simulink model "XTHERM05_reference"  (R2025a)
settings: Solver=daessc  StartTime=0  StopTime=240  MaxStep=1  RelTol=1e-3  AbsTol=1e-3
undefined symbols (not defined in the file): battery_builder_rtmsupport, charge_current_A, charge_step_fraction, charge_step_time_s, coolant_inlet_temperature_K, gcbh, initial_battery_temperature_K
libraries: BatteryPack96S3P_lib x12, fl_lib x8, nesl_utility x5, BatteryCurrentManagement x1, coolingPlateThermal_lib x1
(part 3 of 3)

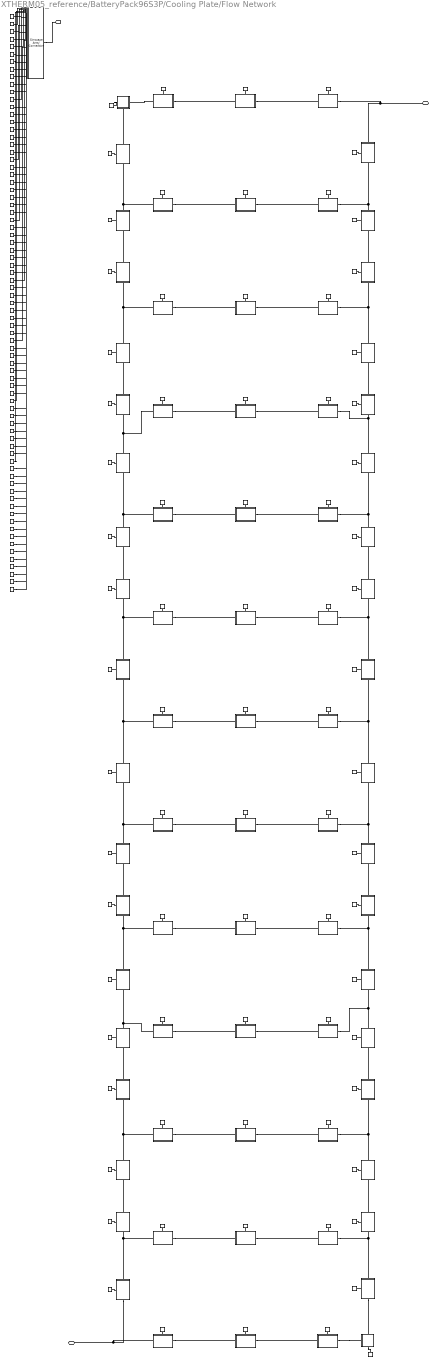
== system XTHERM05_reference/BatteryPack96S3P/Cooling Plate/Flow Network ==
  note: Partition [3,8]
  note: Partition [3,7]
  note: Partition [3,6]
  note: Partition [3,5]
  note: Partition [3,4]
  note: Partition [3,3]
  note: Partition [3,2]
  note: Partition [3,1]
  note: Partition [2,8]
  note: Partition [2,7]
  note: Partition [2,6]
  note: Partition [2,5]
  note: Partition [2,4]
  note: Partition [2,3]
  note: Partition [2,2]
  note: Partition [2,1]
  note: Partition [1,8]
  note: Partition [1,7]
  note: Partition [1,6]
  note: Partition [1,5]
  note: Partition [1,4]
  note: Partition [1,3]
  note: Partition [1,2]
  note: Partition [1,1]
  Array Connection : SimscapeArrayConnection  Domain=foundation.thermal.thermal  NumScalarElements=77
  Bend1_1 : Subsystem  ReferencedSubsystem=BendSubsystemWithMask  lengthPipe=0.0031376  areaPipe=3.1416e-06  diaPipe=0.002  dirPipeOrientBend=up-right
      settings: PortSchema="{\"entries\":[{\"content\":{\"sides\":[{\"content\":{\"connectorIds\":[\"LConn1\"]},\"type\":\"ConnectorPlacement.EquallySpacedRectSide\",\"uuid\":\"fe1e9e2d-1739-4737-8ec3-440461fb646e\"},{\"content\":{\"side\":\"RIGHT\"},\"type\":\"ConnectorPlacement.EquallySpacedRectSide\",\"uuid\":\"c44e4257-eb38-4c5c-b0bd-b7832920e0b4\"},{\"content\":{\"connectorIds\":[\"LConn2\"],\"side\":\"TOP\"},\"type\":\"ConnectorPlacement.EquallySpacedRectSide\",\"uuid\":\"152ce001-782f-4a48-bd0b-9533b0313205\"},{\"content\":{\"connectorIds\":[\"RConn1\"],\"side\":\"BOTTOM\"},\"type\":\"ConnectorPlacement.EquallySpacedRectSide\",\"uuid\":\"9f8ea262-ac4d-418e-a81f-297a07a7dff2\"}]},\"type\":\"ConnectorPlacement.EquallySpacedConnector\",\"uuid\":\"fea8adfe-ce64-4d7f-ba34-bc1e0cac7b5f\"}],\"packageUris\":[\"http://schema.mathworks.com/mf0/Connector/R2020b\"],\"version\":\"1.0\"}"
  Bend2_1 : Subsystem  ReferencedSubsystem=BendSubsystemWithMask  lengthPipe=0.0031376  areaPipe=3.1416e-06  diaPipe=0.002  dirPipeOrientBend=up-right
      settings: PortSchema="{\"entries\":[{\"content\":{\"sides\":[{\"content\":{\"connectorIds\":[\"LConn1\"]},\"type\":\"ConnectorPlacement.EquallySpacedRectSide\",\"uuid\":\"fe1e9e2d-1739-4737-8ec3-440461fb646e\"},{\"content\":{\"side\":\"RIGHT\"},\"type\":\"ConnectorPlacement.EquallySpacedRectSide\",\"uuid\":\"c44e4257-eb38-4c5c-b0bd-b7832920e0b4\"},{\"content\":{\"connectorIds\":[\"LConn2\"],\"side\":\"TOP\"},\"type\":\"ConnectorPlacement.EquallySpacedRectSide\",\"uuid\":\"152ce001-782f-4a48-bd0b-9533b0313205\"},{\"content\":{\"connectorIds\":[\"RConn1\"],\"side\":\"BOTTOM\"},\"type\":\"ConnectorPlacement.EquallySpacedRectSide\",\"uuid\":\"780a4b5e-c251-4558-87ca-52d2b2f91024\"}]},\"type\":\"ConnectorPlacement.EquallySpacedConnector\",\"uuid\":\"fea8adfe-ce64-4d7f-ba34-bc1e0cac7b5f\"}],\"packageUris\":[\"http://schema.mathworks.com/mf0/Connector/R2020b\"],\"version\":\"1.0\"}"
  H_10_1 : ConnectionLabel  Label=H_10_1
  H_10_1_bus : ConnectionLabel  Label=H_10_1
  H_10_2 : ConnectionLabel  Label=H_10_2
  H_10_2_bus : ConnectionLabel  Label=H_10_2
  H_10_3 : ConnectionLabel  Label=H_10_3
  H_10_3_bus : ConnectionLabel  Label=H_10_3
  H_11_1 : ConnectionLabel  Label=H_11_1
  H_11_1_bus : ConnectionLabel  Label=H_11_1
  H_11_2 : ConnectionLabel  Label=H_11_2
  H_11_2_bus : ConnectionLabel  Label=H_11_2
  H_11_3 : ConnectionLabel  Label=H_11_3
  H_11_3_bus : ConnectionLabel  Label=H_11_3
  H_12_1 : ConnectionLabel  Label=H_12_1
  H_12_1_bus : ConnectionLabel  Label=H_12_1
  H_12_2 : ConnectionLabel  Label=H_12_2
  H_12_2_bus : ConnectionLabel  Label=H_12_2
  H_12_3 : ConnectionLabel  Label=H_12_3
  H_12_3_bus : ConnectionLabel  Label=H_12_3
  H_13_1 : ConnectionLabel  Label=H_13_1
  H_13_1_bus : ConnectionLabel  Label=H_13_1
  H_13_2 : ConnectionLabel  Label=H_13_2
  H_13_2_bus : ConnectionLabel  Label=H_13_2
  H_13_3 : ConnectionLabel  Label=H_13_3
  H_13_3_bus : ConnectionLabel  Label=H_13_3
  H_14_1 : ConnectionLabel  Label=H_14_1
  H_14_1_bus : ConnectionLabel  Label=H_14_1
  H_15_1 : ConnectionLabel  Label=H_15_1
  H_15_1_bus : ConnectionLabel  Label=H_15_1
  H_15_2 : ConnectionLabel  Label=H_15_2
  H_15_2_bus : ConnectionLabel  Label=H_15_2
  H_16_1 : ConnectionLabel  Label=H_16_1
  H_16_1_bus : ConnectionLabel  Label=H_16_1
  H_16_2 : ConnectionLabel  Label=H_16_2
  H_16_2_bus : ConnectionLabel  Label=H_16_2
  H_17_1 : ConnectionLabel  Label=H_17_1
  H_17_1_bus : ConnectionLabel  Label=H_17_1
  H_18_1 : ConnectionLabel  Label=H_18_1
  H_18_1_bus : ConnectionLabel  Label=H_18_1
  H_18_2 : ConnectionLabel  Label=H_18_2
  H_18_2_bus : ConnectionLabel  Label=H_18_2
  H_19_1 : ConnectionLabel  Label=H_19_1
  H_19_1_bus : ConnectionLabel  Label=H_19_1
  H_1_1 : ConnectionLabel  Label=H_1_1
  H_1_1_bus : ConnectionLabel  Label=H_1_1
  H_1_2 : ConnectionLabel  Label=H_1_2
  H_1_2_bus : ConnectionLabel  Label=H_1_2
  H_1_3 : ConnectionLabel  Label=H_1_3
  H_1_3_bus : ConnectionLabel  Label=H_1_3
  H_20_1 : ConnectionLabel  Label=H_20_1
  H_20_1_bus : ConnectionLabel  Label=H_20_1
  H_21_1 : ConnectionLabel  Label=H_21_1
  H_21_1_bus : ConnectionLabel  Label=H_21_1
  H_21_2 : ConnectionLabel  Label=H_21_2
  H_21_2_bus : ConnectionLabel  Label=H_21_2
  H_22_1 : ConnectionLabel  Label=H_22_1
  H_22_1_bus : ConnectionLabel  Label=H_22_1
  H_23_1 : ConnectionLabel  Label=H_23_1
  H_23_1_bus : ConnectionLabel  Label=H_23_1
  H_23_2 : ConnectionLabel  Label=H_23_2
  H_23_2_bus : ConnectionLabel  Label=H_23_2
  H_24_1 : ConnectionLabel  Label=H_24_1
  H_24_1_bus : ConnectionLabel  Label=H_24_1
  H_24_2 : ConnectionLabel  Label=H_24_2
  H_24_2_bus : ConnectionLabel  Label=H_24_2
  H_25_1 : ConnectionLabel  Label=H_25_1
  H_25_1_bus : ConnectionLabel  Label=H_25_1
  H_26_1 : ConnectionLabel  Label=H_26_1
  H_26_1_bus : ConnectionLabel  Label=H_26_1
  H_27_1 : ConnectionLabel  Label=H_27_1
  H_27_1_bus : ConnectionLabel  Label=H_27_1
  H_27_2 : ConnectionLabel  Label=H_27_2
  H_27_2_bus : ConnectionLabel  Label=H_27_2
  H_28_1 : ConnectionLabel  Label=H_28_1
  H_28_1_bus : ConnectionLabel  Label=H_28_1
  H_28_2 : ConnectionLabel  Label=H_28_2
  H_28_2_bus : ConnectionLabel  Label=H_28_2
  H_29_1 : ConnectionLabel  Label=H_29_1
  H_29_1_bus : ConnectionLabel  Label=H_29_1
  H_2_1 : ConnectionLabel  Label=H_2_1
  H_2_1_bus : ConnectionLabel  Label=H_2_1
  H_2_2 : ConnectionLabel  Label=H_2_2
  H_2_2_bus : ConnectionLabel  Label=H_2_2
  H_2_3 : ConnectionLabel  Label=H_2_3
  H_2_3_bus : ConnectionLabel  Label=H_2_3
  H_30_1 : ConnectionLabel  Label=H_30_1
  H_30_1_bus : ConnectionLabel  Label=H_30_1
  H_30_2 : ConnectionLabel  Label=H_30_2
  H_30_2_bus : ConnectionLabel  Label=H_30_2
  H_31_1 : ConnectionLabel  Label=H_31_1
  H_31_1_bus : ConnectionLabel  Label=H_31_1
  H_32_1 : ConnectionLabel  Label=H_32_1
  H_32_1_bus : ConnectionLabel  Label=H_32_1
  H_33_1 : ConnectionLabel  Label=H_33_1
  H_33_1_bus : ConnectionLabel  Label=H_33_1
  H_33_2 : ConnectionLabel  Label=H_33_2
  H_33_2_bus : ConnectionLabel  Label=H_33_2
  H_34_1 : ConnectionLabel  Label=H_34_1
  H_34_1_bus : ConnectionLabel  Label=H_34_1
  H_35_1 : ConnectionLabel  Label=H_35_1
  H_35_1_bus : ConnectionLabel  Label=H_35_1
  H_35_2 : ConnectionLabel  Label=H_35_2
  H_35_2_bus : ConnectionLabel  Label=H_35_2
  H_36_1 : ConnectionLabel  Label=H_36_1
  H_36_1_bus : ConnectionLabel  Label=H_36_1
  H_36_2 : ConnectionLabel  Label=H_36_2
  H_36_2_bus : ConnectionLabel  Label=H_36_2
  H_37_1 : ConnectionLabel  Label=H_37_1
  H_37_1_bus : ConnectionLabel  Label=H_37_1
  H_38_1 : ConnectionLabel  Label=H_38_1
  H_38_1_bus : ConnectionLabel  Label=H_38_1
  H_39_1 : ConnectionLabel  Label=H_39_1
  H_39_1_bus : ConnectionLabel  Label=H_39_1
  H_3_1 : ConnectionLabel  Label=H_3_1
  H_3_1_bus : ConnectionLabel  Label=H_3_1
  H_3_2 : ConnectionLabel  Label=H_3_2
  H_3_2_bus : ConnectionLabel  Label=H_3_2
  H_3_3 : ConnectionLabel  Label=H_3_3
  H_3_3_bus : ConnectionLabel  Label=H_3_3
  H_4_1 : ConnectionLabel  Label=H_4_1
  H_4_1_bus : ConnectionLabel  Label=H_4_1
  H_4_2 : ConnectionLabel  Label=H_4_2
  H_4_2_bus : ConnectionLabel  Label=H_4_2
  H_4_3 : ConnectionLabel  Label=H_4_3
  H_4_3_bus : ConnectionLabel  Label=H_4_3
  H_5_1 : ConnectionLabel  Label=H_5_1
  H_5_1_bus : ConnectionLabel  Label=H_5_1
  H_5_2 : ConnectionLabel  Label=H_5_2
  H_5_2_bus : ConnectionLabel  Label=H_5_2
  H_5_3 : ConnectionLabel  Label=H_5_3
  H_5_3_bus : ConnectionLabel  Label=H_5_3
  H_6_1 : ConnectionLabel  Label=H_6_1
  H_6_1_bus : ConnectionLabel  Label=H_6_1
  H_6_2 : ConnectionLabel  Label=H_6_2
  H_6_2_bus : ConnectionLabel  Label=H_6_2
  H_6_3 : ConnectionLabel  Label=H_6_3
  H_6_3_bus : ConnectionLabel  Label=H_6_3
  H_7_1 : ConnectionLabel  Label=H_7_1
  H_7_1_bus : ConnectionLabel  Label=H_7_1
  H_7_2 : ConnectionLabel  Label=H_7_2
  H_7_2_bus : ConnectionLabel  Label=H_7_2
  H_7_3 : ConnectionLabel  Label=H_7_3
  H_7_3_bus : ConnectionLabel  Label=H_7_3
  H_8_1 : ConnectionLabel  Label=H_8_1
  H_8_1_bus : ConnectionLabel  Label=H_8_1
  H_8_2 : ConnectionLabel  Label=H_8_2
  H_8_2_bus : ConnectionLabel  Label=H_8_2
  H_8_3 : ConnectionLabel  Label=H_8_3
  H_8_3_bus : ConnectionLabel  Label=H_8_3
  H_9_1 : ConnectionLabel  Label=H_9_1
  H_9_1_bus : ConnectionLabel  Label=H_9_1
  H_9_2 : ConnectionLabel  Label=H_9_2
  H_9_2_bus : ConnectionLabel  Label=H_9_2
  H_9_3 : ConnectionLabel  Label=H_9_3
  H_9_3_bus : ConnectionLabel  Label=H_9_3
  Pipe10_1 : Subsystem  ReferencedSubsystem=PipeSubsystemWithMask  lengthPipe=0.36667  areaPipe=3.1416e-06  diaPipe=0.002  directionPipe=right
      settings: PortSchema="{\"entries\":[{\"content\":{\"sides\":[{\"content\":{\"connectorIds\":[\"LConn1\"]},\"type\":\"ConnectorPlacement.EquallySpacedRectSide\",\"uuid\":\"fe1e9e2d-1739-4737-8ec3-440461fb646e\"},{\"content\":{\"connectorIds\":[\"RConn1\"],\"side\":\"RIGHT\"},\"type\":\"ConnectorPlacement.EquallySpacedRectSide\",\"uuid\":\"c44e4257-eb38-4c5c-b0bd-b7832920e0b4\"},{\"content\":{\"connectorIds\":[\"LConn2\"],\"side\":\"TOP\"},\"type\":\"ConnectorPlacement.EquallySpacedRectSide\",\"uuid\":\"152ce001-782f-4a48-bd0b-9533b0313205\"}]},\"type\":\"ConnectorPlacement.EquallySpacedConnector\",\"uuid\":\"fea8adfe-ce64-4d7f-ba34-bc1e0cac7b5f\"}],\"packageUris\":[\"http://schema.mathworks.com/mf0/Connector/R2020b\"],\"version\":\"1.0\"}"
  Pipe10_2 : Subsystem  ReferencedSubsystem=PipeSubsystemWithMask  lengthPipe=0.39167  areaPipe=3.1416e-06  diaPipe=0.002  directionPipe=right
      settings: PortSchema="{\"entries\":[{\"content\":{\"sides\":[{\"content\":{\"connectorIds\":[\"LConn1\"]},\"type\":\"ConnectorPlacement.EquallySpacedRectSide\",\"uuid\":\"fe1e9e2d-1739-4737-8ec3-440461fb646e\"},{\"content\":{\"connectorIds\":[\"RConn1\"],\"side\":\"RIGHT\"},\"type\":\"ConnectorPlacement.EquallySpacedRectSide\",\"uuid\":\"c44e4257-eb38-4c5c-b0bd-b7832920e0b4\"},{\"content\":{\"connectorIds\":[\"LConn2\"],\"side\":\"TOP\"},\"type\":\"ConnectorPlacement.EquallySpacedRectSide\",\"uuid\":\"152ce001-782f-4a48-bd0b-9533b0313205\"}]},\"type\":\"ConnectorPlacement.EquallySpacedConnector\",\"uuid\":\"fea8adfe-ce64-4d7f-ba34-bc1e0cac7b5f\"}],\"packageUris\":[\"http://schema.mathworks.com/mf0/Connector/R2020b\"],\"version\":\"1.0\"}"
  Pipe10_3 : Subsystem  ReferencedSubsystem=PipeSubsystemWithMask  lengthPipe=0.36667  areaPipe=3.1416e-06  diaPipe=0.002  directionPipe=right
      settings: PortSchema="{\"entries\":[{\"content\":{\"sides\":[{\"content\":{\"connectorIds\":[\"LConn1\"]},\"type\":\"ConnectorPlacement.EquallySpacedRectSide\",\"uuid\":\"fe1e9e2d-1739-4737-8ec3-440461fb646e\"},{\"content\":{\"connectorIds\":[\"RConn1\"],\"side\":\"RIGHT\"},\"type\":\"ConnectorPlacement.EquallySpacedRectSide\",\"uuid\":\"c44e4257-eb38-4c5c-b0bd-b7832920e0b4\"},{\"content\":{\"connectorIds\":[\"LConn2\"],\"side\":\"TOP\"},\"type\":\"ConnectorPlacement.EquallySpacedRectSide\",\"uuid\":\"152ce001-782f-4a48-bd0b-9533b0313205\"}]},\"type\":\"ConnectorPlacement.EquallySpacedConnector\",\"uuid\":\"fea8adfe-ce64-4d7f-ba34-bc1e0cac7b5f\"}],\"packageUris\":[\"http://schema.mathworks.com/mf0/Connector/R2020b\"],\"version\":\"1.0\"}"
  Pipe11_1 : Subsystem  ReferencedSubsystem=PipeSubsystemWithMask  lengthPipe=0.36667  areaPipe=3.1416e-06  diaPipe=0.002  directionPipe=right
      settings: PortSchema="{\"entries\":[{\"content\":{\"sides\":[{\"content\":{\"connectorIds\":[\"LConn1\"]},\"type\":\"ConnectorPlacement.EquallySpacedRectSide\",\"uuid\":\"fe1e9e2d-1739-4737-8ec3-440461fb646e\"},{\"content\":{\"connectorIds\":[\"RConn1\"],\"side\":\"RIGHT\"},\"type\":\"ConnectorPlacement.EquallySpacedRectSide\",\"uuid\":\"c44e4257-eb38-4c5c-b0bd-b7832920e0b4\"},{\"content\":{\"connectorIds\":[\"LConn2\"],\"side\":\"TOP\"},\"type\":\"ConnectorPlacement.EquallySpacedRectSide\",\"uuid\":\"152ce001-782f-4a48-bd0b-9533b0313205\"}]},\"type\":\"ConnectorPlacement.EquallySpacedConnector\",\"uuid\":\"fea8adfe-ce64-4d7f-ba34-bc1e0cac7b5f\"}],\"packageUris\":[\"http://schema.mathworks.com/mf0/Connector/R2020b\"],\"version\":\"1.0\"}"
  Pipe11_2 : Subsystem  ReferencedSubsystem=PipeSubsystemWithMask  lengthPipe=0.39167  areaPipe=3.1416e-06  diaPipe=0.002  directionPipe=right
      settings: PortSchema="{\"entries\":[{\"content\":{\"sides\":[{\"content\":{\"connectorIds\":[\"LConn1\"]},\"type\":\"ConnectorPlacement.EquallySpacedRectSide\",\"uuid\":\"fe1e9e2d-1739-4737-8ec3-440461fb646e\"},{\"content\":{\"connectorIds\":[\"RConn1\"],\"side\":\"RIGHT\"},\"type\":\"ConnectorPlacement.EquallySpacedRectSide\",\"uuid\":\"c44e4257-eb38-4c5c-b0bd-b7832920e0b4\"},{\"content\":{\"connectorIds\":[\"LConn2\"],\"side\":\"TOP\"},\"type\":\"ConnectorPlacement.EquallySpacedRectSide\",\"uuid\":\"152ce001-782f-4a48-bd0b-9533b0313205\"}]},\"type\":\"ConnectorPlacement.EquallySpacedConnector\",\"uuid\":\"fea8adfe-ce64-4d7f-ba34-bc1e0cac7b5f\"}],\"packageUris\":[\"http://schema.mathworks.com/mf0/Connector/R2020b\"],\"version\":\"1.0\"}"
  Pipe11_3 : Subsystem  ReferencedSubsystem=PipeSubsystemWithMask  lengthPipe=0.36667  areaPipe=3.1416e-06  diaPipe=0.002  directionPipe=right
      settings: PortSchema="{\"entries\":[{\"content\":{\"sides\":[{\"content\":{\"connectorIds\":[\"LConn1\"]},\"type\":\"ConnectorPlacement.EquallySpacedRectSide\",\"uuid\":\"fe1e9e2d-1739-4737-8ec3-440461fb646e\"},{\"content\":{\"connectorIds\":[\"RConn1\"],\"side\":\"RIGHT\"},\"type\":\"ConnectorPlacement.EquallySpacedRectSide\",\"uuid\":\"c44e4257-eb38-4c5c-b0bd-b7832920e0b4\"},{\"content\":{\"connectorIds\":[\"LConn2\"],\"side\":\"TOP\"},\"type\":\"ConnectorPlacement.EquallySpacedRectSide\",\"uuid\":\"152ce001-782f-4a48-bd0b-9533b0313205\"}]},\"type\":\"ConnectorPlacement.EquallySpacedConnector\",\"uuid\":\"fea8adfe-ce64-4d7f-ba34-bc1e0cac7b5f\"}],\"packageUris\":[\"http://schema.mathworks.com/mf0/Connector/R2020b\"],\"version\":\"1.0\"}"
  Pipe12_1 : Subsystem  ReferencedSubsystem=PipeSubsystemWithMask  lengthPipe=0.36667  areaPipe=3.1416e-06  diaPipe=0.002  directionPipe=right
      settings: PortSchema="{\"entries\":[{\"content\":{\"sides\":[{\"content\":{\"connectorIds\":[\"LConn1\"]},\"type\":\"ConnectorPlacement.EquallySpacedRectSide\",\"uuid\":\"fe1e9e2d-1739-4737-8ec3-440461fb646e\"},{\"content\":{\"connectorIds\":[\"RConn1\"],\"side\":\"RIGHT\"},\"type\":\"ConnectorPlacement.EquallySpacedRectSide\",\"uuid\":\"c44e4257-eb38-4c5c-b0bd-b7832920e0b4\"},{\"content\":{\"connectorIds\":[\"LConn2\"],\"side\":\"TOP\"},\"type\":\"ConnectorPlacement.EquallySpacedRectSide\",\"uuid\":\"152ce001-782f-4a48-bd0b-9533b0313205\"}]},\"type\":\"ConnectorPlacement.EquallySpacedConnector\",\"uuid\":\"fea8adfe-ce64-4d7f-ba34-bc1e0cac7b5f\"}],\"packageUris\":[\"http://schema.mathworks.com/mf0/Connector/R2020b\"],\"version\":\"1.0\"}"
  Pipe12_2 : Subsystem  ReferencedSubsystem=PipeSubsystemWithMask  lengthPipe=0.39167  areaPipe=3.1416e-06  diaPipe=0.002  directionPipe=right
      settings: PortSchema="{\"entries\":[{\"content\":{\"sides\":[{\"content\":{\"connectorIds\":[\"LConn1\"]},\"type\":\"ConnectorPlacement.EquallySpacedRectSide\",\"uuid\":\"fe1e9e2d-1739-4737-8ec3-440461fb646e\"},{\"content\":{\"connectorIds\":[\"RConn1\"],\"side\":\"RIGHT\"},\"type\":\"ConnectorPlacement.EquallySpacedRectSide\",\"uuid\":\"c44e4257-eb38-4c5c-b0bd-b7832920e0b4\"},{\"content\":{\"connectorIds\":[\"LConn2\"],\"side\":\"TOP\"},\"type\":\"ConnectorPlacement.EquallySpacedRectSide\",\"uuid\":\"152ce001-782f-4a48-bd0b-9533b0313205\"}]},\"type\":\"ConnectorPlacement.EquallySpacedConnector\",\"uuid\":\"fea8adfe-ce64-4d7f-ba34-bc1e0cac7b5f\"}],\"packageUris\":[\"http://schema.mathworks.com/mf0/Connector/R2020b\"],\"version\":\"1.0\"}"
  Pipe12_3 : Subsystem  ReferencedSubsystem=PipeSubsystemWithMask  lengthPipe=0.36667  areaPipe=3.1416e-06  diaPipe=0.002  directionPipe=right
      settings: PortSchema="{\"entries\":[{\"content\":{\"sides\":[{\"content\":{\"connectorIds\":[\"LConn1\"]},\"type\":\"ConnectorPlacement.EquallySpacedRectSide\",\"uuid\":\"fe1e9e2d-1739-4737-8ec3-440461fb646e\"},{\"content\":{\"connectorIds\":[\"RConn1\"],\"side\":\"RIGHT\"},\"type\":\"ConnectorPlacement.EquallySpacedRectSide\",\"uuid\":\"c44e4257-eb38-4c5c-b0bd-b7832920e0b4\"},{\"content\":{\"connectorIds\":[\"LConn2\"],\"side\":\"TOP\"},\"type\":\"ConnectorPlacement.EquallySpacedRectSide\",\"uuid\":\"152ce001-782f-4a48-bd0b-9533b0313205\"}]},\"type\":\"ConnectorPlacement.EquallySpacedConnector\",\"uuid\":\"fea8adfe-ce64-4d7f-ba34-bc1e0cac7b5f\"}],\"packageUris\":[\"http://schema.mathworks.com/mf0/Connector/R2020b\"],\"version\":\"1.0\"}"
  Pipe13_1 : Subsystem  ReferencedSubsystem=PipeSubsystemWithMask  lengthPipe=0.36467  areaPipe=3.1416e-06  diaPipe=0.002  directionPipe=right
      settings: PortSchema="{\"entries\":[{\"content\":{\"sides\":[{\"content\":{\"connectorIds\":[\"LConn1\"]},\"type\":\"ConnectorPlacement.EquallySpacedRectSide\",\"uuid\":\"fe1e9e2d-1739-4737-8ec3-440461fb646e\"},{\"content\":{\"connectorIds\":[\"RConn1\"],\"side\":\"RIGHT\"},\"type\":\"ConnectorPlacement.EquallySpacedRectSide\",\"uuid\":\"c44e4257-eb38-4c5c-b0bd-b7832920e0b4\"},{\"content\":{\"connectorIds\":[\"LConn2\"],\"side\":\"TOP\"},\"type\":\"ConnectorPlacement.EquallySpacedRectSide\",\"uuid\":\"152ce001-782f-4a48-bd0b-9533b0313205\"}]},\"type\":\"ConnectorPlacement.EquallySpacedConnector\",\"uuid\":\"fea8adfe-ce64-4d7f-ba34-bc1e0cac7b5f\"}],\"packageUris\":[\"http://schema.mathworks.com/mf0/Connector/R2020b\"],\"version\":\"1.0\"}"
  Pipe13_2 : Subsystem  ReferencedSubsystem=PipeSubsystemWithMask  lengthPipe=0.39167  areaPipe=3.1416e-06  diaPipe=0.002  directionPipe=right
      settings: PortSchema="{\"entries\":[{\"content\":{\"sides\":[{\"content\":{\"connectorIds\":[\"LConn1\"]},\"type\":\"ConnectorPlacement.EquallySpacedRectSide\",\"uuid\":\"fe1e9e2d-1739-4737-8ec3-440461fb646e\"},{\"content\":{\"connectorIds\":[\"RConn1\"],\"side\":\"RIGHT\"},\"type\":\"ConnectorPlacement.EquallySpacedRectSide\",\"uuid\":\"c44e4257-eb38-4c5c-b0bd-b7832920e0b4\"},{\"content\":{\"connectorIds\":[\"LConn2\"],\"side\":\"TOP\"},\"type\":\"ConnectorPlacement.EquallySpacedRectSide\",\"uuid\":\"152ce001-782f-4a48-bd0b-9533b0313205\"}]},\"type\":\"ConnectorPlacement.EquallySpacedConnector\",\"uuid\":\"fea8adfe-ce64-4d7f-ba34-bc1e0cac7b5f\"}],\"packageUris\":[\"http://schema.mathworks.com/mf0/Connector/R2020b\"],\"version\":\"1.0\"}"
  Pipe13_3 : Subsystem  ReferencedSubsystem=PipeSubsystemWithMask  lengthPipe=0.36667  areaPipe=3.1416e-06  diaPipe=0.002  directionPipe=right
      settings: PortSchema="{\"entries\":[{\"content\":{\"sides\":[{\"content\":{\"connectorIds\":[\"LConn1\"]},\"type\":\"ConnectorPlacement.EquallySpacedRectSide\",\"uuid\":\"fe1e9e2d-1739-4737-8ec3-440461fb646e\"},{\"content\":{\"connectorIds\":[\"RConn1\"],\"side\":\"RIGHT\"},\"type\":\"ConnectorPlacement.EquallySpacedRectSide\",\"uuid\":\"c44e4257-eb38-4c5c-b0bd-b7832920e0b4\"},{\"content\":{\"connectorIds\":[\"LConn2\"],\"side\":\"TOP\"},\"type\":\"ConnectorPlacement.EquallySpacedRectSide\",\"uuid\":\"152ce001-782f-4a48-bd0b-9533b0313205\"}]},\"type\":\"ConnectorPlacement.EquallySpacedConnector\",\"uuid\":\"fea8adfe-ce64-4d7f-ba34-bc1e0cac7b5f\"}],\"packageUris\":[\"http://schema.mathworks.com/mf0/Connector/R2020b\"],\"version\":\"1.0\"}"
  Pipe14_1 : Subsystem  ReferencedSubsystem=PipeSubsystemWithMask  lengthPipe=0.1  areaPipe=3.1416e-06  diaPipe=0.002  directionPipe=up
      settings: PortSchema="{\"entries\":[{\"content\":{\"sides\":[{\"content\":{\"connectorIds\":[\"LConn1\"]},\"type\":\"ConnectorPlacement.EquallySpacedRectSide\",\"uuid\":\"fe1e9e2d-1739-4737-8ec3-440461fb646e\"},{\"content\":{\"connectorIds\":[\"RConn1\"],\"side\":\"RIGHT\"},\"type\":\"ConnectorPlacement.EquallySpacedRectSide\",\"uuid\":\"c44e4257-eb38-4c5c-b0bd-b7832920e0b4\"},{\"content\":{\"connectorIds\":[\"LConn2\"],\"side\":\"TOP\"},\"type\":\"ConnectorPlacement.EquallySpacedRectSide\",\"uuid\":\"152ce001-782f-4a48-bd0b-9533b0313205\"}]},\"type\":\"ConnectorPlacement.EquallySpacedConnector\",\"uuid\":\"fea8adfe-ce64-4d7f-ba34-bc1e0cac7b5f\"}],\"packageUris\":[\"http://schema.mathworks.com/mf0/Connector/R2020b\"],\"version\":\"1.0\"}"
  Pipe15_1 : Subsystem  ReferencedSubsystem=PipeSubsystemWithMask  lengthPipe=0.03125  areaPipe=3.1416e-06  diaPipe=0.002  directionPipe=up
      settings: PortSchema="{\"entries\":[{\"content\":{\"sides\":[{\"content\":{\"connectorIds\":[\"LConn1\"]},\"type\":\"ConnectorPlacement.EquallySpacedRectSide\",\"uuid\":\"fe1e9e2d-1739-4737-8ec3-440461fb646e\"},{\"content\":{\"connectorIds\":[\"RConn1\"],\"side\":\"RIGHT\"},\"type\":\"ConnectorPlacement.EquallySpacedRectSide\",\"uuid\":\"c44e4257-eb38-4c5c-b0bd-b7832920e0b4\"},{\"content\":{\"connectorIds\":[\"LConn2\"],\"side\":\"TOP\"},\"type\":\"ConnectorPlacement.EquallySpacedRectSide\",\"uuid\":\"152ce001-782f-4a48-bd0b-9533b0313205\"}]},\"type\":\"ConnectorPlacement.EquallySpacedConnector\",\"uuid\":\"fea8adfe-ce64-4d7f-ba34-bc1e0cac7b5f\"}],\"packageUris\":[\"http://schema.mathworks.com/mf0/Connector/R2020b\"],\"version\":\"1.0\"}"
  Pipe15_2 : Subsystem  ReferencedSubsystem=PipeSubsystemWithMask  lengthPipe=0.06875  areaPipe=3.1416e-06  diaPipe=0.002  directionPipe=up
      settings: PortSchema="{\"entries\":[{\"content\":{\"sides\":[{\"content\":{\"connectorIds\":[\"LConn1\"]},\"type\":\"ConnectorPlacement.EquallySpacedRectSide\",\"uuid\":\"fe1e9e2d-1739-4737-8ec3-440461fb646e\"},{\"content\":{\"connectorIds\":[\"RConn1\"],\"side\":\"RIGHT\"},\"type\":\"ConnectorPlacement.EquallySpacedRectSide\",\"uuid\":\"c44e4257-eb38-4c5c-b0bd-b7832920e0b4\"},{\"content\":{\"connectorIds\":[\"LConn2\"],\"side\":\"TOP\"},\"type\":\"ConnectorPlacement.EquallySpacedRectSide\",\"uuid\":\"152ce001-782f-4a48-bd0b-9533b0313205\"}]},\"type\":\"ConnectorPlacement.EquallySpacedConnector\",\"uuid\":\"fea8adfe-ce64-4d7f-ba34-bc1e0cac7b5f\"}],\"packageUris\":[\"http://schema.mathworks.com/mf0/Connector/R2020b\"],\"version\":\"1.0\"}"
  Pipe16_1 : Subsystem  ReferencedSubsystem=PipeSubsystemWithMask  lengthPipe=0.0875  areaPipe=3.1416e-06  diaPipe=0.002  directionPipe=up
      settings: PortSchema="{\"entries\":[{\"content\":{\"sides\":[{\"content\":{\"connectorIds\":[\"LConn1\"]},\"type\":\"ConnectorPlacement.EquallySpacedRectSide\",\"uuid\":\"fe1e9e2d-1739-4737-8ec3-440461fb646e\"},{\"content\":{\"connectorIds\":[\"RConn1\"],\"side\":\"RIGHT\"},\"type\":\"ConnectorPlacement.EquallySpacedRectSide\",\"uuid\":\"c44e4257-eb38-4c5c-b0bd-b7832920e0b4\"},{\"content\":{\"connectorIds\":[\"LConn2\"],\"side\":\"TOP\"},\"type\":\"ConnectorPlacement.EquallySpacedRectSide\",\"uuid\":\"152ce001-782f-4a48-bd0b-9533b0313205\"}]},\"type\":\"ConnectorPlacement.EquallySpacedConnector\",\"uuid\":\"fea8adfe-ce64-4d7f-ba34-bc1e0cac7b5f\"}],\"packageUris\":[\"http://schema.mathworks.com/mf0/Connector/R2020b\"],\"version\":\"1.0\"}"
  Pipe16_2 : Subsystem  ReferencedSubsystem=PipeSubsystemWithMask  lengthPipe=0.0125  areaPipe=3.1416e-06  diaPipe=0.002  directionPipe=up
      settings: PortSchema="{\"entries\":[{\"content\":{\"sides\":[{\"content\":{\"connectorIds\":[\"LConn1\"]},\"type\":\"ConnectorPlacement.EquallySpacedRectSide\",\"uuid\":\"fe1e9e2d-1739-4737-8ec3-440461fb646e\"},{\"content\":{\"connectorIds\":[\"RConn1\"],\"side\":\"RIGHT\"},\"type\":\"ConnectorPlacement.EquallySpacedRectSide\",\"uuid\":\"c44e4257-eb38-4c5c-b0bd-b7832920e0b4\"},{\"content\":{\"connectorIds\":[\"LConn2\"],\"side\":\"TOP\"},\"type\":\"ConnectorPlacement.EquallySpacedRectSide\",\"uuid\":\"152ce001-782f-4a48-bd0b-9533b0313205\"}]},\"type\":\"ConnectorPlacement.EquallySpacedConnector\",\"uuid\":\"fea8adfe-ce64-4d7f-ba34-bc1e0cac7b5f\"}],\"packageUris\":[\"http://schema.mathworks.com/mf0/Connector/R2020b\"],\"version\":\"1.0\"}"
  Pipe17_1 : Subsystem  ReferencedSubsystem=PipeSubsystemWithMask  lengthPipe=0.1  areaPipe=3.1416e-06  diaPipe=0.002  directionPipe=up
      settings: PortSchema="{\"entries\":[{\"content\":{\"sides\":[{\"content\":{\"connectorIds\":[\"LConn1\"]},\"type\":\"ConnectorPlacement.EquallySpacedRectSide\",\"uuid\":\"fe1e9e2d-1739-4737-8ec3-440461fb646e\"},{\"content\":{\"connectorIds\":[\"RConn1\"],\"side\":\"RIGHT\"},\"type\":\"ConnectorPlacement.EquallySpacedRectSide\",\"uuid\":\"c44e4257-eb38-4c5c-b0bd-b7832920e0b4\"},{\"content\":{\"connectorIds\":[\"LConn2\"],\"side\":\"TOP\"},\"type\":\"ConnectorPlacement.EquallySpacedRectSide\",\"uuid\":\"152ce001-782f-4a48-bd0b-9533b0313205\"}]},\"type\":\"ConnectorPlacement.EquallySpacedConnector\",\"uuid\":\"fea8adfe-ce64-4d7f-ba34-bc1e0cac7b5f\"}],\"packageUris\":[\"http://schema.mathworks.com/mf0/Connector/R2020b\"],\"version\":\"1.0\"}"
  Pipe18_1 : Subsystem  ReferencedSubsystem=PipeSubsystemWithMask  lengthPipe=0.04375  areaPipe=3.1416e-06  diaPipe=0.002  directionPipe=up
      settings: PortSchema="{\"entries\":[{\"content\":{\"sides\":[{\"content\":{\"connectorIds\":[\"LConn1\"]},\"type\":\"ConnectorPlacement.EquallySpacedRectSide\",\"uuid\":\"fe1e9e2d-1739-4737-8ec3-440461fb646e\"},{\"content\":{\"connectorIds\":[\"RConn1\"],\"side\":\"RIGHT\"},\"type\":\"ConnectorPlacement.EquallySpacedRectSide\",\"uuid\":\"c44e4257-eb38-4c5c-b0bd-b7832920e0b4\"},{\"content\":{\"connectorIds\":[\"LConn2\"],\"side\":\"TOP\"},\"type\":\"ConnectorPlacement.EquallySpacedRectSide\",\"uuid\":\"152ce001-782f-4a48-bd0b-9533b0313205\"}]},\"type\":\"ConnectorPlacement.EquallySpacedConnector\",\"uuid\":\"fea8adfe-ce64-4d7f-ba34-bc1e0cac7b5f\"}],\"packageUris\":[\"http://schema.mathworks.com/mf0/Connector/R2020b\"],\"version\":\"1.0\"}"
  Pipe18_2 : Subsystem  ReferencedSubsystem=PipeSubsystemWithMask  lengthPipe=0.05625  areaPipe=3.1416e-06  diaPipe=0.002  directionPipe=up
      settings: PortSchema="{\"entries\":[{\"content\":{\"sides\":[{\"content\":{\"connectorIds\":[\"LConn1\"]},\"type\":\"ConnectorPlacement.EquallySpacedRectSide\",\"uuid\":\"fe1e9e2d-1739-4737-8ec3-440461fb646e\"},{\"content\":{\"connectorIds\":[\"RConn1\"],\"side\":\"RIGHT\"},\"type\":\"ConnectorPlacement.EquallySpacedRectSide\",\"uuid\":\"c44e4257-eb38-4c5c-b0bd-b7832920e0b4\"},{\"content\":{\"connectorIds\":[\"LConn2\"],\"side\":\"TOP\"},\"type\":\"ConnectorPlacement.EquallySpacedRectSide\",\"uuid\":\"152ce001-782f-4a48-bd0b-9533b0313205\"}]},\"type\":\"ConnectorPlacement.EquallySpacedConnector\",\"uuid\":\"fea8adfe-ce64-4d7f-ba34-bc1e0cac7b5f\"}],\"packageUris\":[\"http://schema.mathworks.com/mf0/Connector/R2020b\"],\"version\":\"1.0\"}"
  Pipe19_1 : Subsystem  ReferencedSubsystem=PipeSubsystemWithMask  lengthPipe=0.1  areaPipe=3.1416e-06  diaPipe=0.002  directionPipe=up
      settings: PortSchema="{\"entries\":[{\"content\":{\"sides\":[{\"content\":{\"connectorIds\":[\"LConn1\"]},\"type\":\"ConnectorPlacement.EquallySpacedRectSide\",\"uuid\":\"fe1e9e2d-1739-4737-8ec3-440461fb646e\"},{\"content\":{\"connectorIds\":[\"RConn1\"],\"side\":\"RIGHT\"},\"type\":\"ConnectorPlacement.EquallySpacedRectSide\",\"uuid\":\"c44e4257-eb38-4c5c-b0bd-b7832920e0b4\"},{\"content\":{\"connectorIds\":[\"LConn2\"],\"side\":\"TOP\"},\"type\":\"ConnectorPlacement.EquallySpacedRectSide\",\"uuid\":\"152ce001-782f-4a48-bd0b-9533b0313205\"}]},\"type\":\"ConnectorPlacement.EquallySpacedConnector\",\"uuid\":\"fea8adfe-ce64-4d7f-ba34-bc1e0cac7b5f\"}],\"packageUris\":[\"http://schema.mathworks.com/mf0/Connector/R2020b\"],\"version\":\"1.0\"}"
  Pipe1_1 : Subsystem  ReferencedSubsystem=PipeSubsystemWithMask  lengthPipe=0.36667  areaPipe=3.1416e-06  diaPipe=0.002  directionPipe=right
      settings: PortSchema="{\"entries\":[{\"content\":{\"sides\":[{\"content\":{\"connectorIds\":[\"LConn1\"]},\"type\":\"ConnectorPlacement.EquallySpacedRectSide\",\"uuid\":\"fe1e9e2d-1739-4737-8ec3-440461fb646e\"},{\"content\":{\"connectorIds\":[\"RConn1\"],\"side\":\"RIGHT\"},\"type\":\"ConnectorPlacement.EquallySpacedRectSide\",\"uuid\":\"c44e4257-eb38-4c5c-b0bd-b7832920e0b4\"},{\"content\":{\"connectorIds\":[\"LConn2\"],\"side\":\"TOP\"},\"type\":\"ConnectorPlacement.EquallySpacedRectSide\",\"uuid\":\"152ce001-782f-4a48-bd0b-9533b0313205\"}]},\"type\":\"ConnectorPlacement.EquallySpacedConnector\",\"uuid\":\"fea8adfe-ce64-4d7f-ba34-bc1e0cac7b5f\"}],\"packageUris\":[\"http://schema.mathworks.com/mf0/Connector/R2020b\"],\"version\":\"1.0\"}"
  Pipe1_2 : Subsystem  ReferencedSubsystem=PipeSubsystemWithMask  lengthPipe=0.39167  areaPipe=3.1416e-06  diaPipe=0.002  directionPipe=right
      settings: PortSchema="{\"entries\":[{\"content\":{\"sides\":[{\"content\":{\"connectorIds\":[\"LConn1\"]},\"type\":\"ConnectorPlacement.EquallySpacedRectSide\",\"uuid\":\"fe1e9e2d-1739-4737-8ec3-440461fb646e\"},{\"content\":{\"connectorIds\":[\"RConn1\"],\"side\":\"RIGHT\"},\"type\":\"ConnectorPlacement.EquallySpacedRectSide\",\"uuid\":\"c44e4257-eb38-4c5c-b0bd-b7832920e0b4\"},{\"content\":{\"connectorIds\":[\"LConn2\"],\"side\":\"TOP\"},\"type\":\"ConnectorPlacement.EquallySpacedRectSide\",\"uuid\":\"152ce001-782f-4a48-bd0b-9533b0313205\"}]},\"type\":\"ConnectorPlacement.EquallySpacedConnector\",\"uuid\":\"fea8adfe-ce64-4d7f-ba34-bc1e0cac7b5f\"}],\"packageUris\":[\"http://schema.mathworks.com/mf0/Connector/R2020b\"],\"version\":\"1.0\"}"
  Pipe1_3 : Subsystem  ReferencedSubsystem=PipeSubsystemWithMask  lengthPipe=0.36467  areaPipe=3.1416e-06  diaPipe=0.002  directionPipe=right
      settings: PortSchema="{\"entries\":[{\"content\":{\"sides\":[{\"content\":{\"connectorIds\":[\"LConn1\"]},\"type\":\"ConnectorPlacement.EquallySpacedRectSide\",\"uuid\":\"fe1e9e2d-1739-4737-8ec3-440461fb646e\"},{\"content\":{\"connectorIds\":[\"RConn1\"],\"side\":\"RIGHT\"},\"type\":\"ConnectorPlacement.EquallySpacedRectSide\",\"uuid\":\"c44e4257-eb38-4c5c-b0bd-b7832920e0b4\"},{\"content\":{\"connectorIds\":[\"LConn2\"],\"side\":\"TOP\"},\"type\":\"ConnectorPlacement.EquallySpacedRectSide\",\"uuid\":\"152ce001-782f-4a48-bd0b-9533b0313205\"}]},\"type\":\"ConnectorPlacement.EquallySpacedConnector\",\"uuid\":\"fea8adfe-ce64-4d7f-ba34-bc1e0cac7b5f\"}],\"packageUris\":[\"http://schema.mathworks.com/mf0/Connector/R2020b\"],\"version\":\"1.0\"}"
  Pipe20_1 : Subsystem  ReferencedSubsystem=PipeSubsystemWithMask  lengthPipe=0.1  areaPipe=3.1416e-06  diaPipe=0.002  directionPipe=up
      settings: PortSchema="{\"entries\":[{\"content\":{\"sides\":[{\"content\":{\"connectorIds\":[\"LConn1\"]},\"type\":\"ConnectorPlacement.EquallySpacedRectSide\",\"uuid\":\"fe1e9e2d-1739-4737-8ec3-440461fb646e\"},{\"content\":{\"connectorIds\":[\"RConn1\"],\"side\":\"RIGHT\"},\"type\":\"ConnectorPlacement.EquallySpacedRectSide\",\"uuid\":\"c44e4257-eb38-4c5c-b0bd-b7832920e0b4\"},{\"content\":{\"connectorIds\":[\"LConn2\"],\"side\":\"TOP\"},\"type\":\"ConnectorPlacement.EquallySpacedRectSide\",\"uuid\":\"152ce001-782f-4a48-bd0b-9533b0313205\"}]},\"type\":\"ConnectorPlacement.EquallySpacedConnector\",\"uuid\":\"fea8adfe-ce64-4d7f-ba34-bc1e0cac7b5f\"}],\"packageUris\":[\"http://schema.mathworks.com/mf0/Connector/R2020b\"],\"version\":\"1.0\"}"
  Pipe21_1 : Subsystem  ReferencedSubsystem=PipeSubsystemWithMask  lengthPipe=0.05625  areaPipe=3.1416e-06  diaPipe=0.002  directionPipe=up
      settings: PortSchema="{\"entries\":[{\"content\":{\"sides\":[{\"content\":{\"connectorIds\":[\"LConn1\"]},\"type\":\"ConnectorPlacement.EquallySpacedRectSide\",\"uuid\":\"fe1e9e2d-1739-4737-8ec3-440461fb646e\"},{\"content\":{\"connectorIds\":[\"RConn1\"],\"side\":\"RIGHT\"},\"type\":\"ConnectorPlacement.EquallySpacedRectSide\",\"uuid\":\"c44e4257-eb38-4c5c-b0bd-b7832920e0b4\"},{\"content\":{\"connectorIds\":[\"LConn2\"],\"side\":\"TOP\"},\"type\":\"ConnectorPlacement.EquallySpacedRectSide\",\"uuid\":\"152ce001-782f-4a48-bd0b-9533b0313205\"}]},\"type\":\"ConnectorPlacement.EquallySpacedConnector\",\"uuid\":\"fea8adfe-ce64-4d7f-ba34-bc1e0cac7b5f\"}],\"packageUris\":[\"http://schema.mathworks.com/mf0/Connector/R2020b\"],\"version\":\"1.0\"}"
  Pipe21_2 : Subsystem  ReferencedSubsystem=PipeSubsystemWithMask  lengthPipe=0.04375  areaPipe=3.1416e-06  diaPipe=0.002  directionPipe=up
      settings: PortSchema="{\"entries\":[{\"content\":{\"sides\":[{\"content\":{\"connectorIds\":[\"LConn1\"]},\"type\":\"ConnectorPlacement.EquallySpacedRectSide\",\"uuid\":\"fe1e9e2d-1739-4737-8ec3-440461fb646e\"},{\"content\":{\"connectorIds\":[\"RConn1\"],\"side\":\"RIGHT\"},\"type\":\"ConnectorPlacement.EquallySpacedRectSide\",\"uuid\":\"c44e4257-eb38-4c5c-b0bd-b7832920e0b4\"},{\"content\":{\"connectorIds\":[\"LConn2\"],\"side\":\"TOP\"},\"type\":\"ConnectorPlacement.EquallySpacedRectSide\",\"uuid\":\"152ce001-782f-4a48-bd0b-9533b0313205\"}]},\"type\":\"ConnectorPlacement.EquallySpacedConnector\",\"uuid\":\"fea8adfe-ce64-4d7f-ba34-bc1e0cac7b5f\"}],\"packageUris\":[\"http://schema.mathworks.com/mf0/Connector/R2020b\"],\"version\":\"1.0\"}"
  Pipe22_1 : Subsystem  ReferencedSubsystem=PipeSubsystemWithMask  lengthPipe=0.1  areaPipe=3.1416e-06  diaPipe=0.002  directionPipe=up
      settings: PortSchema="{\"entries\":[{\"content\":{\"sides\":[{\"content\":{\"connectorIds\":[\"LConn1\"]},\"type\":\"ConnectorPlacement.EquallySpacedRectSide\",\"uuid\":\"fe1e9e2d-1739-4737-8ec3-440461fb646e\"},{\"content\":{\"connectorIds\":[\"RConn1\"],\"side\":\"RIGHT\"},\"type\":\"ConnectorPlacement.EquallySpacedRectSide\",\"uuid\":\"c44e4257-eb38-4c5c-b0bd-b7832920e0b4\"},{\"content\":{\"connectorIds\":[\"LConn2\"],\"side\":\"TOP\"},\"type\":\"ConnectorPlacement.EquallySpacedRectSide\",\"uuid\":\"152ce001-782f-4a48-bd0b-9533b0313205\"}]},\"type\":\"ConnectorPlacement.EquallySpacedConnector\",\"uuid\":\"fea8adfe-ce64-4d7f-ba34-bc1e0cac7b5f\"}],\"packageUris\":[\"http://schema.mathworks.com/mf0/Connector/R2020b\"],\"version\":\"1.0\"}"
  Pipe23_1 : Subsystem  ReferencedSubsystem=PipeSubsystemWithMask  lengthPipe=0.0125  areaPipe=3.1416e-06  diaPipe=0.002  directionPipe=up
      settings: PortSchema="{\"entries\":[{\"content\":{\"sides\":[{\"content\":{\"connectorIds\":[\"LConn1\"]},\"type\":\"ConnectorPlacement.EquallySpacedRectSide\",\"uuid\":\"fe1e9e2d-1739-4737-8ec3-440461fb646e\"},{\"content\":{\"connectorIds\":[\"RConn1\"],\"side\":\"RIGHT\"},\"type\":\"ConnectorPlacement.EquallySpacedRectSide\",\"uuid\":\"c44e4257-eb38-4c5c-b0bd-b7832920e0b4\"},{\"content\":{\"connectorIds\":[\"LConn2\"],\"side\":\"TOP\"},\"type\":\"ConnectorPlacement.EquallySpacedRectSide\",\"uuid\":\"152ce001-782f-4a48-bd0b-9533b0313205\"}]},\"type\":\"ConnectorPlacement.EquallySpacedConnector\",\"uuid\":\"fea8adfe-ce64-4d7f-ba34-bc1e0cac7b5f\"}],\"packageUris\":[\"http://schema.mathworks.com/mf0/Connector/R2020b\"],\"version\":\"1.0\"}"
  Pipe23_2 : Subsystem  ReferencedSubsystem=PipeSubsystemWithMask  lengthPipe=0.0875  areaPipe=3.1416e-06  diaPipe=0.002  directionPipe=up
      settings: PortSchema="{\"entries\":[{\"content\":{\"sides\":[{\"content\":{\"connectorIds\":[\"LConn1\"]},\"type\":\"ConnectorPlacement.EquallySpacedRectSide\",\"uuid\":\"fe1e9e2d-1739-4737-8ec3-440461fb646e\"},{\"content\":{\"connectorIds\":[\"RConn1\"],\"side\":\"RIGHT\"},\"type\":\"ConnectorPlacement.EquallySpacedRectSide\",\"uuid\":\"c44e4257-eb38-4c5c-b0bd-b7832920e0b4\"},{\"content\":{\"connectorIds\":[\"LConn2\"],\"side\":\"TOP\"},\"type\":\"ConnectorPlacement.EquallySpacedRectSide\",\"uuid\":\"152ce001-782f-4a48-bd0b-9533b0313205\"}]},\"type\":\"ConnectorPlacement.EquallySpacedConnector\",\"uuid\":\"fea8adfe-ce64-4d7f-ba34-bc1e0cac7b5f\"}],\"packageUris\":[\"http://schema.mathworks.com/mf0/Connector/R2020b\"],\"version\":\"1.0\"}"
  Pipe24_1 : Subsystem  ReferencedSubsystem=PipeSubsystemWithMask  lengthPipe=0.06875  areaPipe=3.1416e-06  diaPipe=0.002  directionPipe=up
      settings: PortSchema="{\"entries\":[{\"content\":{\"sides\":[{\"content\":{\"connectorIds\":[\"LConn1\"]},\"type\":\"ConnectorPlacement.EquallySpacedRectSide\",\"uuid\":\"fe1e9e2d-1739-4737-8ec3-440461fb646e\"},{\"content\":{\"connectorIds\":[\"RConn1\"],\"side\":\"RIGHT\"},\"type\":\"ConnectorPlacement.EquallySpacedRectSide\",\"uuid\":\"c44e4257-eb38-4c5c-b0bd-b7832920e0b4\"},{\"content\":{\"connectorIds\":[\"LConn2\"],\"side\":\"TOP\"},\"type\":\"ConnectorPlacement.EquallySpacedRectSide\",\"uuid\":\"152ce001-782f-4a48-bd0b-9533b0313205\"}]},\"type\":\"ConnectorPlacement.EquallySpacedConnector\",\"uuid\":\"fea8adfe-ce64-4d7f-ba34-bc1e0cac7b5f\"}],\"packageUris\":[\"http://schema.mathworks.com/mf0/Connector/R2020b\"],\"version\":\"1.0\"}"
  Pipe24_2 : Subsystem  ReferencedSubsystem=PipeSubsystemWithMask  lengthPipe=0.03125  areaPipe=3.1416e-06  diaPipe=0.002  directionPipe=up
      settings: PortSchema="{\"entries\":[{\"content\":{\"sides\":[{\"content\":{\"connectorIds\":[\"LConn1\"]},\"type\":\"ConnectorPlacement.EquallySpacedRectSide\",\"uuid\":\"fe1e9e2d-1739-4737-8ec3-440461fb646e\"},{\"content\":{\"connectorIds\":[\"RConn1\"],\"side\":\"RIGHT\"},\"type\":\"ConnectorPlacement.EquallySpacedRectSide\",\"uuid\":\"c44e4257-eb38-4c5c-b0bd-b7832920e0b4\"},{\"content\":{\"connectorIds\":[\"LConn2\"],\"side\":\"TOP\"},\"type\":\"ConnectorPlacement.EquallySpacedRectSide\",\"uuid\":\"152ce001-782f-4a48-bd0b-9533b0313205\"}]},\"type\":\"ConnectorPlacement.EquallySpacedConnector\",\"uuid\":\"fea8adfe-ce64-4d7f-ba34-bc1e0cac7b5f\"}],\"packageUris\":[\"http://schema.mathworks.com/mf0/Connector/R2020b\"],\"version\":\"1.0\"}"
  Pipe25_1 : Subsystem  ReferencedSubsystem=PipeSubsystemWithMask  lengthPipe=0.098  areaPipe=3.1416e-06  diaPipe=0.002  directionPipe=up
      settings: PortSchema="{\"entries\":[{\"content\":{\"sides\":[{\"content\":{\"connectorIds\":[\"LConn1\"]},\"type\":\"ConnectorPlacement.EquallySpacedRectSide\",\"uuid\":\"fe1e9e2d-1739-4737-8ec3-440461fb646e\"},{\"content\":{\"connectorIds\":[\"RConn1\"],\"side\":\"RIGHT\"},\"type\":\"ConnectorPlacement.EquallySpacedRectSide\",\"uuid\":\"c44e4257-eb38-4c5c-b0bd-b7832920e0b4\"},{\"content\":{\"connectorIds\":[\"LConn2\"],\"side\":\"TOP\"},\"type\":\"ConnectorPlacement.EquallySpacedRectSide\",\"uuid\":\"152ce001-782f-4a48-bd0b-9533b0313205\"}]},\"type\":\"ConnectorPlacement.EquallySpacedConnector\",\"uuid\":\"fea8adfe-ce64-4d7f-ba34-bc1e0cac7b5f\"}],\"packageUris\":[\"http://schema.mathworks.com/mf0/Connector/R2020b\"],\"version\":\"1.0\"}"
  Pipe26_1 : Subsystem  ReferencedSubsystem=PipeSubsystemWithMask  lengthPipe=0.098  areaPipe=3.1416e-06  diaPipe=0.002  directionPipe=up
      settings: PortSchema="{\"entries\":[{\"content\":{\"sides\":[{\"content\":{\"connectorIds\":[\"LConn1\"]},\"type\":\"ConnectorPlacement.EquallySpacedRectSide\",\"uuid\":\"fe1e9e2d-1739-4737-8ec3-440461fb646e\"},{\"content\":{\"connectorIds\":[\"RConn1\"],\"side\":\"RIGHT\"},\"type\":\"ConnectorPlacement.EquallySpacedRectSide\",\"uuid\":\"c44e4257-eb38-4c5c-b0bd-b7832920e0b4\"},{\"content\":{\"connectorIds\":[\"LConn2\"],\"side\":\"TOP\"},\"type\":\"ConnectorPlacement.EquallySpacedRectSide\",\"uuid\":\"152ce001-782f-4a48-bd0b-9533b0313205\"}]},\"type\":\"ConnectorPlacement.EquallySpacedConnector\",\"uuid\":\"fea8adfe-ce64-4d7f-ba34-bc1e0cac7b5f\"}],\"packageUris\":[\"http://schema.mathworks.com/mf0/Connector/R2020b\"],\"version\":\"1.0\"}"
  Pipe27_1 : Subsystem  ReferencedSubsystem=PipeSubsystemWithMask  lengthPipe=0.03125  areaPipe=3.1416e-06  diaPipe=0.002  directionPipe=up
      settings: PortSchema="{\"entries\":[{\"content\":{\"sides\":[{\"content\":{\"connectorIds\":[\"LConn1\"]},\"type\":\"ConnectorPlacement.EquallySpacedRectSide\",\"uuid\":\"fe1e9e2d-1739-4737-8ec3-440461fb646e\"},{\"content\":{\"connectorIds\":[\"RConn1\"],\"side\":\"RIGHT\"},\"type\":\"ConnectorPlacement.EquallySpacedRectSide\",\"uuid\":\"c44e4257-eb38-4c5c-b0bd-b7832920e0b4\"},{\"content\":{\"connectorIds\":[\"LConn2\"],\"side\":\"TOP\"},\"type\":\"ConnectorPlacement.EquallySpacedRectSide\",\"uuid\":\"152ce001-782f-4a48-bd0b-9533b0313205\"}]},\"type\":\"ConnectorPlacement.EquallySpacedConnector\",\"uuid\":\"fea8adfe-ce64-4d7f-ba34-bc1e0cac7b5f\"}],\"packageUris\":[\"http://schema.mathworks.com/mf0/Connector/R2020b\"],\"version\":\"1.0\"}"
  Pipe27_2 : Subsystem  ReferencedSubsystem=PipeSubsystemWithMask  lengthPipe=0.06875  areaPipe=3.1416e-06  diaPipe=0.002  directionPipe=up
      settings: PortSchema="{\"entries\":[{\"content\":{\"sides\":[{\"content\":{\"connectorIds\":[\"LConn1\"]},\"type\":\"ConnectorPlacement.EquallySpacedRectSide\",\"uuid\":\"fe1e9e2d-1739-4737-8ec3-440461fb646e\"},{\"content\":{\"connectorIds\":[\"RConn1\"],\"side\":\"RIGHT\"},\"type\":\"ConnectorPlacement.EquallySpacedRectSide\",\"uuid\":\"c44e4257-eb38-4c5c-b0bd-b7832920e0b4\"},{\"content\":{\"connectorIds\":[\"LConn2\"],\"side\":\"TOP\"},\"type\":\"ConnectorPlacement.EquallySpacedRectSide\",\"uuid\":\"152ce001-782f-4a48-bd0b-9533b0313205\"}]},\"type\":\"ConnectorPlacement.EquallySpacedConnector\",\"uuid\":\"fea8adfe-ce64-4d7f-ba34-bc1e0cac7b5f\"}],\"packageUris\":[\"http://schema.mathworks.com/mf0/Connector/R2020b\"],\"version\":\"1.0\"}"
  Pipe28_1 : Subsystem  ReferencedSubsystem=PipeSubsystemWithMask  lengthPipe=0.0875  areaPipe=3.1416e-06  diaPipe=0.002  directionPipe=up
      settings: PortSchema="{\"entries\":[{\"content\":{\"sides\":[{\"content\":{\"connectorIds\":[\"LConn1\"]},\"type\":\"ConnectorPlacement.EquallySpacedRectSide\",\"uuid\":\"fe1e9e2d-1739-4737-8ec3-440461fb646e\"},{\"content\":{\"connectorIds\":[\"RConn1\"],\"side\":\"RIGHT\"},\"type\":\"ConnectorPlacement.EquallySpacedRectSide\",\"uuid\":\"c44e4257-eb38-4c5c-b0bd-b7832920e0b4\"},{\"content\":{\"connectorIds\":[\"LConn2\"],\"side\":\"TOP\"},\"type\":\"ConnectorPlacement.EquallySpacedRectSide\",\"uuid\":\"152ce001-782f-4a48-bd0b-9533b0313205\"}]},\"type\":\"ConnectorPlacement.EquallySpacedConnector\",\"uuid\":\"fea8adfe-ce64-4d7f-ba34-bc1e0cac7b5f\"}],\"packageUris\":[\"http://schema.mathworks.com/mf0/Connector/R2020b\"],\"version\":\"1.0\"}"
  Pipe28_2 : Subsystem  ReferencedSubsystem=PipeSubsystemWithMask  lengthPipe=0.0125  areaPipe=3.1416e-06  diaPipe=0.002  directionPipe=up
      settings: PortSchema="{\"entries\":[{\"content\":{\"sides\":[{\"content\":{\"connectorIds\":[\"LConn1\"]},\"type\":\"ConnectorPlacement.EquallySpacedRectSide\",\"uuid\":\"fe1e9e2d-1739-4737-8ec3-440461fb646e\"},{\"content\":{\"connectorIds\":[\"RConn1\"],\"side\":\"RIGHT\"},\"type\":\"ConnectorPlacement.EquallySpacedRectSide\",\"uuid\":\"c44e4257-eb38-4c5c-b0bd-b7832920e0b4\"},{\"content\":{\"connectorIds\":[\"LConn2\"],\"side\":\"TOP\"},\"type\":\"ConnectorPlacement.EquallySpacedRectSide\",\"uuid\":\"152ce001-782f-4a48-bd0b-9533b0313205\"}]},\"type\":\"ConnectorPlacement.EquallySpacedConnector\",\"uuid\":\"fea8adfe-ce64-4d7f-ba34-bc1e0cac7b5f\"}],\"packageUris\":[\"http://schema.mathworks.com/mf0/Connector/R2020b\"],\"version\":\"1.0\"}"
  Pipe29_1 : Subsystem  ReferencedSubsystem=PipeSubsystemWithMask  lengthPipe=0.1  areaPipe=3.1416e-06  diaPipe=0.002  directionPipe=up
      settings: PortSchema="{\"entries\":[{\"content\":{\"sides\":[{\"content\":{\"connectorIds\":[\"LConn1\"]},\"type\":\"ConnectorPlacement.EquallySpacedRectSide\",\"uuid\":\"fe1e9e2d-1739-4737-8ec3-440461fb646e\"},{\"content\":{\"connectorIds\":[\"RConn1\"],\"side\":\"RIGHT\"},\"type\":\"ConnectorPlacement.EquallySpacedRectSide\",\"uuid\":\"c44e4257-eb38-4c5c-b0bd-b7832920e0b4\"},{\"content\":{\"connectorIds\":[\"LConn2\"],\"side\":\"TOP\"},\"type\":\"ConnectorPlacement.EquallySpacedRectSide\",\"uuid\":\"152ce001-782f-4a48-bd0b-9533b0313205\"}]},\"type\":\"ConnectorPlacement.EquallySpacedConnector\",\"uuid\":\"fea8adfe-ce64-4d7f-ba34-bc1e0cac7b5f\"}],\"packageUris\":[\"http://schema.mathworks.com/mf0/Connector/R2020b\"],\"version\":\"1.0\"}"
  Pipe2_1 : Subsystem  ReferencedSubsystem=PipeSubsystemWithMask  lengthPipe=0.36667  areaPipe=3.1416e-06  diaPipe=0.002  directionPipe=right
      settings: PortSchema="{\"entries\":[{\"content\":{\"sides\":[{\"content\":{\"connectorIds\":[\"LConn1\"]},\"type\":\"ConnectorPlacement.EquallySpacedRectSide\",\"uuid\":\"fe1e9e2d-1739-4737-8ec3-440461fb646e\"},{\"content\":{\"connectorIds\":[\"RConn1\"],\"side\":\"RIGHT\"},\"type\":\"ConnectorPlacement.EquallySpacedRectSide\",\"uuid\":\"c44e4257-eb38-4c5c-b0bd-b7832920e0b4\"},{\"content\":{\"connectorIds\":[\"LConn2\"],\"side\":\"TOP\"},\"type\":\"ConnectorPlacement.EquallySpacedRectSide\",\"uuid\":\"152ce001-782f-4a48-bd0b-9533b0313205\"}]},\"type\":\"ConnectorPlacement.EquallySpacedConnector\",\"uuid\":\"fea8adfe-ce64-4d7f-ba34-bc1e0cac7b5f\"}],\"packageUris\":[\"http://schema.mathworks.com/mf0/Connector/R2020b\"],\"version\":\"1.0\"}"
  Pipe2_2 : Subsystem  ReferencedSubsystem=PipeSubsystemWithMask  lengthPipe=0.39167  areaPipe=3.1416e-06  diaPipe=0.002  directionPipe=right
      settings: PortSchema="{\"entries\":[{\"content\":{\"sides\":[{\"content\":{\"connectorIds\":[\"LConn1\"]},\"type\":\"ConnectorPlacement.EquallySpacedRectSide\",\"uuid\":\"fe1e9e2d-1739-4737-8ec3-440461fb646e\"},{\"content\":{\"connectorIds\":[\"RConn1\"],\"side\":\"RIGHT\"},\"type\":\"ConnectorPlacement.EquallySpacedRectSide\",\"uuid\":\"c44e4257-eb38-4c5c-b0bd-b7832920e0b4\"},{\"content\":{\"connectorIds\":[\"LConn2\"],\"side\":\"TOP\"},\"type\":\"ConnectorPlacement.EquallySpacedRectSide\",\"uuid\":\"152ce001-782f-4a48-bd0b-9533b0313205\"}]},\"type\":\"ConnectorPlacement.EquallySpacedConnector\",\"uuid\":\"fea8adfe-ce64-4d7f-ba34-bc1e0cac7b5f\"}],\"packageUris\":[\"http://schema.mathworks.com/mf0/Connector/R2020b\"],\"version\":\"1.0\"}"
  Pipe2_3 : Subsystem  ReferencedSubsystem=PipeSubsystemWithMask  lengthPipe=0.36667  areaPipe=3.1416e-06  diaPipe=0.002  directionPipe=right
      settings: PortSchema="{\"entries\":[{\"content\":{\"sides\":[{\"content\":{\"connectorIds\":[\"LConn1\"]},\"type\":\"ConnectorPlacement.EquallySpacedRectSide\",\"uuid\":\"fe1e9e2d-1739-4737-8ec3-440461fb646e\"},{\"content\":{\"connectorIds\":[\"RConn1\"],\"side\":\"RIGHT\"},\"type\":\"ConnectorPlacement.EquallySpacedRectSide\",\"uuid\":\"c44e4257-eb38-4c5c-b0bd-b7832920e0b4\"},{\"content\":{\"connectorIds\":[\"LConn2\"],\"side\":\"TOP\"},\"type\":\"ConnectorPlacement.EquallySpacedRectSide\",\"uuid\":\"152ce001-782f-4a48-bd0b-9533b0313205\"}]},\"type\":\"ConnectorPlacement.EquallySpacedConnector\",\"uuid\":\"fea8adfe-ce64-4d7f-ba34-bc1e0cac7b5f\"}],\"packageUris\":[\"http://schema.mathworks.com/mf0/Connector/R2020b\"],\"version\":\"1.0\"}"
  Pipe30_1 : Subsystem  ReferencedSubsystem=PipeSubsystemWithMask  lengthPipe=0.04375  areaPipe=3.1416e-06  diaPipe=0.002  directionPipe=up
      settings: PortSchema="{\"entries\":[{\"content\":{\"sides\":[{\"content\":{\"connectorIds\":[\"LConn1\"]},\"type\":\"ConnectorPlacement.EquallySpacedRectSide\",\"uuid\":\"fe1e9e2d-1739-4737-8ec3-440461fb646e\"},{\"content\":{\"connectorIds\":[\"RConn1\"],\"side\":\"RIGHT\"},\"type\":\"ConnectorPlacement.EquallySpacedRectSide\",\"uuid\":\"c44e4257-eb38-4c5c-b0bd-b7832920e0b4\"},{\"content\":{\"connectorIds\":[\"LConn2\"],\"side\":\"TOP\"},\"type\":\"ConnectorPlacement.EquallySpacedRectSide\",\"uuid\":\"152ce001-782f-4a48-bd0b-9533b0313205\"}]},\"type\":\"ConnectorPlacement.EquallySpacedConnector\",\"uuid\":\"fea8adfe-ce64-4d7f-ba34-bc1e0cac7b5f\"}],\"packageUris\":[\"http://schema.mathworks.com/mf0/Connector/R2020b\"],\"version\":\"1.0\"}"
  Pipe30_2 : Subsystem  ReferencedSubsystem=PipeSubsystemWithMask  lengthPipe=0.05625  areaPipe=3.1416e-06  diaPipe=0.002  directionPipe=up
      settings: PortSchema="{\"entries\":[{\"content\":{\"sides\":[{\"content\":{\"connectorIds\":[\"LConn1\"]},\"type\":\"ConnectorPlacement.EquallySpacedRectSide\",\"uuid\":\"fe1e9e2d-1739-4737-8ec3-440461fb646e\"},{\"content\":{\"connectorIds\":[\"RConn1\"],\"side\":\"RIGHT\"},\"type\":\"ConnectorPlacement.EquallySpacedRectSide\",\"uuid\":\"c44e4257-eb38-4c5c-b0bd-b7832920e0b4\"},{\"content\":{\"connectorIds\":[\"LConn2\"],\"side\":\"TOP\"},\"type\":\"ConnectorPlacement.EquallySpacedRectSide\",\"uuid\":\"152ce001-782f-4a48-bd0b-9533b0313205\"}]},\"type\":\"ConnectorPlacement.EquallySpacedConnector\",\"uuid\":\"fea8adfe-ce64-4d7f-ba34-bc1e0cac7b5f\"}],\"packageUris\":[\"http://schema.mathworks.com/mf0/Connector/R2020b\"],\"version\":\"1.0\"}"
  Pipe31_1 : Subsystem  ReferencedSubsystem=PipeSubsystemWithMask  lengthPipe=0.1  areaPipe=3.1416e-06  diaPipe=0.002  directionPipe=up
      settings: PortSchema="{\"entries\":[{\"content\":{\"sides\":[{\"content\":{\"connectorIds\":[\"LConn1\"]},\"type\":\"ConnectorPlacement.EquallySpacedRectSide\",\"uuid\":\"fe1e9e2d-1739-4737-8ec3-440461fb646e\"},{\"content\":{\"connectorIds\":[\"RConn1\"],\"side\":\"RIGHT\"},\"type\":\"ConnectorPlacement.EquallySpacedRectSide\",\"uuid\":\"c44e4257-eb38-4c5c-b0bd-b7832920e0b4\"},{\"content\":{\"connectorIds\":[\"LConn2\"],\"side\":\"TOP\"},\"type\":\"ConnectorPlacement.EquallySpacedRectSide\",\"uuid\":\"152ce001-782f-4a48-bd0b-9533b0313205\"}]},\"type\":\"ConnectorPlacement.EquallySpacedConnector\",\"uuid\":\"fea8adfe-ce64-4d7f-ba34-bc1e0cac7b5f\"}],\"packageUris\":[\"http://schema.mathworks.com/mf0/Connector/R2020b\"],\"version\":\"1.0\"}"
  Pipe32_1 : Subsystem  ReferencedSubsystem=PipeSubsystemWithMask  lengthPipe=0.1  areaPipe=3.1416e-06  diaPipe=0.002  directionPipe=up
      settings: PortSchema="{\"entries\":[{\"content\":{\"sides\":[{\"content\":{\"connectorIds\":[\"LConn1\"]},\"type\":\"ConnectorPlacement.EquallySpacedRectSide\",\"uuid\":\"fe1e9e2d-1739-4737-8ec3-440461fb646e\"},{\"content\":{\"connectorIds\":[\"RConn1\"],\"side\":\"RIGHT\"},\"type\":\"ConnectorPlacement.EquallySpacedRectSide\",\"uuid\":\"c44e4257-eb38-4c5c-b0bd-b7832920e0b4\"},{\"content\":{\"connectorIds\":[\"LConn2\"],\"side\":\"TOP\"},\"type\":\"ConnectorPlacement.EquallySpacedRectSide\",\"uuid\":\"152ce001-782f-4a48-bd0b-9533b0313205\"}]},\"type\":\"ConnectorPlacement.EquallySpacedConnector\",\"uuid\":\"fea8adfe-ce64-4d7f-ba34-bc1e0cac7b5f\"}],\"packageUris\":[\"http://schema.mathworks.com/mf0/Connector/R2020b\"],\"version\":\"1.0\"}"
  Pipe33_1 : Subsystem  ReferencedSubsystem=PipeSubsystemWithMask  lengthPipe=0.05625  areaPipe=3.1416e-06  diaPipe=0.002  directionPipe=up
      settings: PortSchema="{\"entries\":[{\"content\":{\"sides\":[{\"content\":{\"connectorIds\":[\"LConn1\"]},\"type\":\"ConnectorPlacement.EquallySpacedRectSide\",\"uuid\":\"fe1e9e2d-1739-4737-8ec3-440461fb646e\"},{\"content\":{\"connectorIds\":[\"RConn1\"],\"side\":\"RIGHT\"},\"type\":\"ConnectorPlacement.EquallySpacedRectSide\",\"uuid\":\"c44e4257-eb38-4c5c-b0bd-b7832920e0b4\"},{\"content\":{\"connectorIds\":[\"LConn2\"],\"side\":\"TOP\"},\"type\":\"ConnectorPlacement.EquallySpacedRectSide\",\"uuid\":\"152ce001-782f-4a48-bd0b-9533b0313205\"}]},\"type\":\"ConnectorPlacement.EquallySpacedConnector\",\"uuid\":\"fea8adfe-ce64-4d7f-ba34-bc1e0cac7b5f\"}],\"packageUris\":[\"http://schema.mathworks.com/mf0/Connector/R2020b\"],\"version\":\"1.0\"}"
  Pipe33_2 : Subsystem  ReferencedSubsystem=PipeSubsystemWithMask  lengthPipe=0.04375  areaPipe=3.1416e-06  diaPipe=0.002  directionPipe=up
      settings: PortSchema="{\"entries\":[{\"content\":{\"sides\":[{\"content\":{\"connectorIds\":[\"LConn1\"]},\"type\":\"ConnectorPlacement.EquallySpacedRectSide\",\"uuid\":\"fe1e9e2d-1739-4737-8ec3-440461fb646e\"},{\"content\":{\"connectorIds\":[\"RConn1\"],\"side\":\"RIGHT\"},\"type\":\"ConnectorPlacement.EquallySpacedRectSide\",\"uuid\":\"c44e4257-eb38-4c5c-b0bd-b7832920e0b4\"},{\"content\":{\"connectorIds\":[\"LConn2\"],\"side\":\"TOP\"},\"type\":\"ConnectorPlacement.EquallySpacedRectSide\",\"uuid\":\"152ce001-782f-4a48-bd0b-9533b0313205\"}]},\"type\":\"ConnectorPlacement.EquallySpacedConnector\",\"uuid\":\"fea8adfe-ce64-4d7f-ba34-bc1e0cac7b5f\"}],\"packageUris\":[\"http://schema.mathworks.com/mf0/Connector/R2020b\"],\"version\":\"1.0\"}"
  Pipe34_1 : Subsystem  ReferencedSubsystem=PipeSubsystemWithMask  lengthPipe=0.1  areaPipe=3.1416e-06  diaPipe=0.002  directionPipe=up
      settings: PortSchema="{\"entries\":[{\"content\":{\"sides\":[{\"content\":{\"connectorIds\":[\"LConn1\"]},\"type\":\"ConnectorPlacement.EquallySpacedRectSide\",\"uuid\":\"fe1e9e2d-1739-4737-8ec3-440461fb646e\"},{\"content\":{\"connectorIds\":[\"RConn1\"],\"side\":\"RIGHT\"},\"type\":\"ConnectorPlacement.EquallySpacedRectSide\",\"uuid\":\"c44e4257-eb38-4c5c-b0bd-b7832920e0b4\"},{\"content\":{\"connectorIds\":[\"LConn2\"],\"side\":\"TOP\"},\"type\":\"ConnectorPlacement.EquallySpacedRectSide\",\"uuid\":\"152ce001-782f-4a48-bd0b-9533b0313205\"}]},\"type\":\"ConnectorPlacement.EquallySpacedConnector\",\"uuid\":\"fea8adfe-ce64-4d7f-ba34-bc1e0cac7b5f\"}],\"packageUris\":[\"http://schema.mathworks.com/mf0/Connector/R2020b\"],\"version\":\"1.0\"}"
  Pipe35_1 : Subsystem  ReferencedSubsystem=PipeSubsystemWithMask  lengthPipe=0.0125  areaPipe=3.1416e-06  diaPipe=0.002  directionPipe=up
      settings: PortSchema="{\"entries\":[{\"content\":{\"sides\":[{\"content\":{\"connectorIds\":[\"LConn1\"]},\"type\":\"ConnectorPlacement.EquallySpacedRectSide\",\"uuid\":\"fe1e9e2d-1739-4737-8ec3-440461fb646e\"},{\"content\":{\"connectorIds\":[\"RConn1\"],\"side\":\"RIGHT\"},\"type\":\"ConnectorPlacement.EquallySpacedRectSide\",\"uuid\":\"c44e4257-eb38-4c5c-b0bd-b7832920e0b4\"},{\"content\":{\"connectorIds\":[\"LConn2\"],\"side\":\"TOP\"},\"type\":\"ConnectorPlacement.EquallySpacedRectSide\",\"uuid\":\"152ce001-782f-4a48-bd0b-9533b0313205\"}]},\"type\":\"ConnectorPlacement.EquallySpacedConnector\",\"uuid\":\"fea8adfe-ce64-4d7f-ba34-bc1e0cac7b5f\"}],\"packageUris\":[\"http://schema.mathworks.com/mf0/Connector/R2020b\"],\"version\":\"1.0\"}"
  Pipe35_2 : Subsystem  ReferencedSubsystem=PipeSubsystemWithMask  lengthPipe=0.0875  areaPipe=3.1416e-06  diaPipe=0.002  directionPipe=up
      settings: PortSchema="{\"entries\":[{\"content\":{\"sides\":[{\"content\":{\"connectorIds\":[\"LConn1\"]},\"type\":\"ConnectorPlacement.EquallySpacedRectSide\",\"uuid\":\"fe1e9e2d-1739-4737-8ec3-440461fb646e\"},{\"content\":{\"connectorIds\":[\"RConn1\"],\"side\":\"RIGHT\"},\"type\":\"ConnectorPlacement.EquallySpacedRectSide\",\"uuid\":\"c44e4257-eb38-4c5c-b0bd-b7832920e0b4\"},{\"content\":{\"connectorIds\":[\"LConn2\"],\"side\":\"TOP\"},\"type\":\"ConnectorPlacement.EquallySpacedRectSide\",\"uuid\":\"152ce001-782f-4a48-bd0b-9533b0313205\"}]},\"type\":\"ConnectorPlacement.EquallySpacedConnector\",\"uuid\":\"fea8adfe-ce64-4d7f-ba34-bc1e0cac7b5f\"}],\"packageUris\":[\"http://schema.mathworks.com/mf0/Connector/R2020b\"],\"version\":\"1.0\"}"
  Pipe36_1 : Subsystem  ReferencedSubsystem=PipeSubsystemWithMask  lengthPipe=0.06875  areaPipe=3.1416e-06  diaPipe=0.002  directionPipe=up
      settings: PortSchema="{\"entries\":[{\"content\":{\"sides\":[{\"content\":{\"connectorIds\":[\"LConn1\"]},\"type\":\"ConnectorPlacement.EquallySpacedRectSide\",\"uuid\":\"fe1e9e2d-1739-4737-8ec3-440461fb646e\"},{\"content\":{\"connectorIds\":[\"RConn1\"],\"side\":\"RIGHT\"},\"type\":\"ConnectorPlacement.EquallySpacedRectSide\",\"uuid\":\"c44e4257-eb38-4c5c-b0bd-b7832920e0b4\"},{\"content\":{\"connectorIds\":[\"LConn2\"],\"side\":\"TOP\"},\"type\":\"ConnectorPlacement.EquallySpacedRectSide\",\"uuid\":\"152ce001-782f-4a48-bd0b-9533b0313205\"}]},\"type\":\"ConnectorPlacement.EquallySpacedConnector\",\"uuid\":\"fea8adfe-ce64-4d7f-ba34-bc1e0cac7b5f\"}],\"packageUris\":[\"http://schema.mathworks.com/mf0/Connector/R2020b\"],\"version\":\"1.0\"}"
  Pipe36_2 : Subsystem  ReferencedSubsystem=PipeSubsystemWithMask  lengthPipe=0.03125  areaPipe=3.1416e-06  diaPipe=0.002  directionPipe=up
      settings: PortSchema="{\"entries\":[{\"content\":{\"sides\":[{\"content\":{\"connectorIds\":[\"LConn1\"]},\"type\":\"ConnectorPlacement.EquallySpacedRectSide\",\"uuid\":\"fe1e9e2d-1739-4737-8ec3-440461fb646e\"},{\"content\":{\"connectorIds\":[\"RConn1\"],\"side\":\"RIGHT\"},\"type\":\"ConnectorPlacement.EquallySpacedRectSide\",\"uuid\":\"c44e4257-eb38-4c5c-b0bd-b7832920e0b4\"},{\"content\":{\"connectorIds\":[\"LConn2\"],\"side\":\"TOP\"},\"type\":\"ConnectorPlacement.EquallySpacedRectSide\",\"uuid\":\"152ce001-782f-4a48-bd0b-9533b0313205\"}]},\"type\":\"ConnectorPlacement.EquallySpacedConnector\",\"uuid\":\"fea8adfe-ce64-4d7f-ba34-bc1e0cac7b5f\"}],\"packageUris\":[\"http://schema.mathworks.com/mf0/Connector/R2020b\"],\"version\":\"1.0\"}"
  Pipe37_1 : Subsystem  ReferencedSubsystem=PipeSubsystemWithMask  lengthPipe=0.1  areaPipe=3.1416e-06  diaPipe=0.002  directionPipe=up
      settings: PortSchema="{\"entries\":[{\"content\":{\"sides\":[{\"content\":{\"connectorIds\":[\"LConn1\"]},\"type\":\"ConnectorPlacement.EquallySpacedRectSide\",\"uuid\":\"fe1e9e2d-1739-4737-8ec3-440461fb646e\"},{\"content\":{\"connectorIds\":[\"RConn1\"],\"side\":\"RIGHT\"},\"type\":\"ConnectorPlacement.EquallySpacedRectSide\",\"uuid\":\"c44e4257-eb38-4c5c-b0bd-b7832920e0b4\"},{\"content\":{\"connectorIds\":[\"LConn2\"],\"side\":\"TOP\"},\"type\":\"ConnectorPlacement.EquallySpacedRectSide\",\"uuid\":\"152ce001-782f-4a48-bd0b-9533b0313205\"}]},\"type\":\"ConnectorPlacement.EquallySpacedConnector\",\"uuid\":\"fea8adfe-ce64-4d7f-ba34-bc1e0cac7b5f\"}],\"packageUris\":[\"http://schema.mathworks.com/mf0/Connector/R2020b\"],\"version\":\"1.0\"}"
  Pipe3_1 : Subsystem  ReferencedSubsystem=PipeSubsystemWithMask  lengthPipe=0.36667  areaPipe=3.1416e-06  diaPipe=0.002  directionPipe=right
      settings: PortSchema="{\"entries\":[{\"content\":{\"sides\":[{\"content\":{\"connectorIds\":[\"LConn1\"]},\"type\":\"ConnectorPlacement.EquallySpacedRectSide\",\"uuid\":\"fe1e9e2d-1739-4737-8ec3-440461fb646e\"},{\"content\":{\"connectorIds\":[\"RConn1\"],\"side\":\"RIGHT\"},\"type\":\"ConnectorPlacement.EquallySpacedRectSide\",\"uuid\":\"c44e4257-eb38-4c5c-b0bd-b7832920e0b4\"},{\"content\":{\"connectorIds\":[\"LConn2\"],\"side\":\"TOP\"},\"type\":\"ConnectorPlacement.EquallySpacedRectSide\",\"uuid\":\"152ce001-782f-4a48-bd0b-9533b0313205\"}]},\"type\":\"ConnectorPlacement.EquallySpacedConnector\",\"uuid\":\"fea8adfe-ce64-4d7f-ba34-bc1e0cac7b5f\"}],\"packageUris\":[\"http://schema.mathworks.com/mf0/Connector/R2020b\"],\"version\":\"1.0\"}"
  Pipe3_2 : Subsystem  ReferencedSubsystem=PipeSubsystemWithMask  lengthPipe=0.39167  areaPipe=3.1416e-06  diaPipe=0.002  directionPipe=right
      settings: PortSchema="{\"entries\":[{\"content\":{\"sides\":[{\"content\":{\"connectorIds\":[\"LConn1\"]},\"type\":\"ConnectorPlacement.EquallySpacedRectSide\",\"uuid\":\"fe1e9e2d-1739-4737-8ec3-440461fb646e\"},{\"content\":{\"connectorIds\":[\"RConn1\"],\"side\":\"RIGHT\"},\"type\":\"ConnectorPlacement.EquallySpacedRectSide\",\"uuid\":\"c44e4257-eb38-4c5c-b0bd-b7832920e0b4\"},{\"content\":{\"connectorIds\":[\"LConn2\"],\"side\":\"TOP\"},\"type\":\"ConnectorPlacement.EquallySpacedRectSide\",\"uuid\":\"152ce001-782f-4a48-bd0b-9533b0313205\"}]},\"type\":\"ConnectorPlacement.EquallySpacedConnector\",\"uuid\":\"fea8adfe-ce64-4d7f-ba34-bc1e0cac7b5f\"}],\"packageUris\":[\"http://schema.mathworks.com/mf0/Connector/R2020b\"],\"version\":\"1.0\"}"
  Pipe3_3 : Subsystem  ReferencedSubsystem=PipeSubsystemWithMask  lengthPipe=0.36667  areaPipe=3.1416e-06  diaPipe=0.002  directionPipe=right
      settings: PortSchema="{\"entries\":[{\"content\":{\"sides\":[{\"content\":{\"connectorIds\":[\"LConn1\"]},\"type\":\"ConnectorPlacement.EquallySpacedRectSide\",\"uuid\":\"fe1e9e2d-1739-4737-8ec3-440461fb646e\"},{\"content\":{\"connectorIds\":[\"RConn1\"],\"side\":\"RIGHT\"},\"type\":\"ConnectorPlacement.EquallySpacedRectSide\",\"uuid\":\"c44e4257-eb38-4c5c-b0bd-b7832920e0b4\"},{\"content\":{\"connectorIds\":[\"LConn2\"],\"side\":\"TOP\"},\"type\":\"ConnectorPlacement.EquallySpacedRectSide\",\"uuid\":\"152ce001-782f-4a48-bd0b-9533b0313205\"}]},\"type\":\"ConnectorPlacement.EquallySpacedConnector\",\"uuid\":\"fea8adfe-ce64-4d7f-ba34-bc1e0cac7b5f\"}],\"packageUris\":[\"http://schema.mathworks.com/mf0/Connector/R2020b\"],\"version\":\"1.0\"}"
  Pipe4_1 : Subsystem  ReferencedSubsystem=PipeSubsystemWithMask  lengthPipe=0.36667  areaPipe=3.1416e-06  diaPipe=0.002  directionPipe=right
      settings: PortSchema="{\"entries\":[{\"content\":{\"sides\":[{\"content\":{\"connectorIds\":[\"LConn1\"]},\"type\":\"ConnectorPlacement.EquallySpacedRectSide\",\"uuid\":\"fe1e9e2d-1739-4737-8ec3-440461fb646e\"},{\"content\":{\"connectorIds\":[\"RConn1\"],\"side\":\"RIGHT\"},\"type\":\"ConnectorPlacement.EquallySpacedRectSide\",\"uuid\":\"c44e4257-eb38-4c5c-b0bd-b7832920e0b4\"},{\"content\":{\"connectorIds\":[\"LConn2\"],\"side\":\"TOP\"},\"type\":\"ConnectorPlacement.EquallySpacedRectSide\",\"uuid\":\"152ce001-782f-4a48-bd0b-9533b0313205\"}]},\"type\":\"ConnectorPlacement.EquallySpacedConnector\",\"uuid\":\"fea8adfe-ce64-4d7f-ba34-bc1e0cac7b5f\"}],\"packageUris\":[\"http://schema.mathworks.com/mf0/Connector/R2020b\"],\"version\":\"1.0\"}"
  Pipe4_2 : Subsystem  ReferencedSubsystem=PipeSubsystemWithMask  lengthPipe=0.39167  areaPipe=3.1416e-06  diaPipe=0.002  directionPipe=right
      settings: PortSchema="{\"entries\":[{\"content\":{\"sides\":[{\"content\":{\"connectorIds\":[\"LConn1\"]},\"type\":\"ConnectorPlacement.EquallySpacedRectSide\",\"uuid\":\"fe1e9e2d-1739-4737-8ec3-440461fb646e\"},{\"content\":{\"connectorIds\":[\"RConn1\"],\"side\":\"RIGHT\"},\"type\":\"ConnectorPlacement.EquallySpacedRectSide\",\"uuid\":\"c44e4257-eb38-4c5c-b0bd-b7832920e0b4\"},{\"content\":{\"connectorIds\":[\"LConn2\"],\"side\":\"TOP\"},\"type\":\"ConnectorPlacement.EquallySpacedRectSide\",\"uuid\":\"152ce001-782f-4a48-bd0b-9533b0313205\"}]},\"type\":\"ConnectorPlacement.EquallySpacedConnector\",\"uuid\":\"fea8adfe-ce64-4d7f-ba34-bc1e0cac7b5f\"}],\"packageUris\":[\"http://schema.mathworks.com/mf0/Connector/R2020b\"],\"version\":\"1.0\"}"
  Pipe4_3 : Subsystem  ReferencedSubsystem=PipeSubsystemWithMask  lengthPipe=0.36667  areaPipe=3.1416e-06  diaPipe=0.002  directionPipe=right
      settings: PortSchema="{\"entries\":[{\"content\":{\"sides\":[{\"content\":{\"connectorIds\":[\"LConn1\"]},\"type\":\"ConnectorPlacement.EquallySpacedRectSide\",\"uuid\":\"fe1e9e2d-1739-4737-8ec3-440461fb646e\"},{\"content\":{\"connectorIds\":[\"RConn1\"],\"side\":\"RIGHT\"},\"type\":\"ConnectorPlacement.EquallySpacedRectSide\",\"uuid\":\"c44e4257-eb38-4c5c-b0bd-b7832920e0b4\"},{\"content\":{\"connectorIds\":[\"LConn2\"],\"side\":\"TOP\"},\"type\":\"ConnectorPlacement.EquallySpacedRectSide\",\"uuid\":\"152ce001-782f-4a48-bd0b-9533b0313205\"}]},\"type\":\"ConnectorPlacement.EquallySpacedConnector\",\"uuid\":\"fea8adfe-ce64-4d7f-ba34-bc1e0cac7b5f\"}],\"packageUris\":[\"http://schema.mathworks.com/mf0/Connector/R2020b\"],\"version\":\"1.0\"}"
  Pipe5_1 : Subsystem  ReferencedSubsystem=PipeSubsystemWithMask  lengthPipe=0.36667  areaPipe=3.1416e-06  diaPipe=0.002  directionPipe=right
      settings: PortSchema="{\"entries\":[{\"content\":{\"sides\":[{\"content\":{\"connectorIds\":[\"LConn1\"]},\"type\":\"ConnectorPlacement.EquallySpacedRectSide\",\"uuid\":\"fe1e9e2d-1739-4737-8ec3-440461fb646e\"},{\"content\":{\"connectorIds\":[\"RConn1\"],\"side\":\"RIGHT\"},\"type\":\"ConnectorPlacement.EquallySpacedRectSide\",\"uuid\":\"c44e4257-eb38-4c5c-b0bd-b7832920e0b4\"},{\"content\":{\"connectorIds\":[\"LConn2\"],\"side\":\"TOP\"},\"type\":\"ConnectorPlacement.EquallySpacedRectSide\",\"uuid\":\"152ce001-782f-4a48-bd0b-9533b0313205\"}]},\"type\":\"ConnectorPlacement.EquallySpacedConnector\",\"uuid\":\"fea8adfe-ce64-4d7f-ba34-bc1e0cac7b5f\"}],\"packageUris\":[\"http://schema.mathworks.com/mf0/Connector/R2020b\"],\"version\":\"1.0\"}"
  Pipe5_2 : Subsystem  ReferencedSubsystem=PipeSubsystemWithMask  lengthPipe=0.39167  areaPipe=3.1416e-06  diaPipe=0.002  directionPipe=right
      settings: PortSchema="{\"entries\":[{\"content\":{\"sides\":[{\"content\":{\"connectorIds\":[\"LConn1\"]},\"type\":\"ConnectorPlacement.EquallySpacedRectSide\",\"uuid\":\"fe1e9e2d-1739-4737-8ec3-440461fb646e\"},{\"content\":{\"connectorIds\":[\"RConn1\"],\"side\":\"RIGHT\"},\"type\":\"ConnectorPlacement.EquallySpacedRectSide\",\"uuid\":\"c44e4257-eb38-4c5c-b0bd-b7832920e0b4\"},{\"content\":{\"connectorIds\":[\"LConn2\"],\"side\":\"TOP\"},\"type\":\"ConnectorPlacement.EquallySpacedRectSide\",\"uuid\":\"152ce001-782f-4a48-bd0b-9533b0313205\"}]},\"type\":\"ConnectorPlacement.EquallySpacedConnector\",\"uuid\":\"fea8adfe-ce64-4d7f-ba34-bc1e0cac7b5f\"}],\"packageUris\":[\"http://schema.mathworks.com/mf0/Connector/R2020b\"],\"version\":\"1.0\"}"
  Pipe5_3 : Subsystem  ReferencedSubsystem=PipeSubsystemWithMask  lengthPipe=0.36667  areaPipe=3.1416e-06  diaPipe=0.002  directionPipe=right
      settings: PortSchema="{\"entries\":[{\"content\":{\"sides\":[{\"content\":{\"connectorIds\":[\"LConn1\"]},\"type\":\"ConnectorPlacement.EquallySpacedRectSide\",\"uuid\":\"fe1e9e2d-1739-4737-8ec3-440461fb646e\"},{\"content\":{\"connectorIds\":[\"RConn1\"],\"side\":\"RIGHT\"},\"type\":\"ConnectorPlacement.EquallySpacedRectSide\",\"uuid\":\"c44e4257-eb38-4c5c-b0bd-b7832920e0b4\"},{\"content\":{\"connectorIds\":[\"LConn2\"],\"side\":\"TOP\"},\"type\":\"ConnectorPlacement.EquallySpacedRectSide\",\"uuid\":\"152ce001-782f-4a48-bd0b-9533b0313205\"}]},\"type\":\"ConnectorPlacement.EquallySpacedConnector\",\"uuid\":\"fea8adfe-ce64-4d7f-ba34-bc1e0cac7b5f\"}],\"packageUris\":[\"http://schema.mathworks.com/mf0/Connector/R2020b\"],\"version\":\"1.0\"}"
  Pipe6_1 : Subsystem  ReferencedSubsystem=PipeSubsystemWithMask  lengthPipe=0.36667  areaPipe=3.1416e-06  diaPipe=0.002  directionPipe=right
      settings: PortSchema="{\"entries\":[{\"content\":{\"sides\":[{\"content\":{\"connectorIds\":[\"LConn1\"]},\"type\":\"ConnectorPlacement.EquallySpacedRectSide\",\"uuid\":\"fe1e9e2d-1739-4737-8ec3-440461fb646e\"},{\"content\":{\"connectorIds\":[\"RConn1\"],\"side\":\"RIGHT\"},\"type\":\"ConnectorPlacement.EquallySpacedRectSide\",\"uuid\":\"c44e4257-eb38-4c5c-b0bd-b7832920e0b4\"},{\"content\":{\"connectorIds\":[\"LConn2\"],\"side\":\"TOP\"},\"type\":\"ConnectorPlacement.EquallySpacedRectSide\",\"uuid\":\"152ce001-782f-4a48-bd0b-9533b0313205\"}]},\"type\":\"ConnectorPlacement.EquallySpacedConnector\",\"uuid\":\"fea8adfe-ce64-4d7f-ba34-bc1e0cac7b5f\"}],\"packageUris\":[\"http://schema.mathworks.com/mf0/Connector/R2020b\"],\"version\":\"1.0\"}"
  Pipe6_2 : Subsystem  ReferencedSubsystem=PipeSubsystemWithMask  lengthPipe=0.39167  areaPipe=3.1416e-06  diaPipe=0.002  directionPipe=right
      settings: PortSchema="{\"entries\":[{\"content\":{\"sides\":[{\"content\":{\"connectorIds\":[\"LConn1\"]},\"type\":\"ConnectorPlacement.EquallySpacedRectSide\",\"uuid\":\"fe1e9e2d-1739-4737-8ec3-440461fb646e\"},{\"content\":{\"connectorIds\":[\"RConn1\"],\"side\":\"RIGHT\"},\"type\":\"ConnectorPlacement.EquallySpacedRectSide\",\"uuid\":\"c44e4257-eb38-4c5c-b0bd-b7832920e0b4\"},{\"content\":{\"connectorIds\":[\"LConn2\"],\"side\":\"TOP\"},\"type\":\"ConnectorPlacement.EquallySpacedRectSide\",\"uuid\":\"152ce001-782f-4a48-bd0b-9533b0313205\"}]},\"type\":\"ConnectorPlacement.EquallySpacedConnector\",\"uuid\":\"fea8adfe-ce64-4d7f-ba34-bc1e0cac7b5f\"}],\"packageUris\":[\"http://schema.mathworks.com/mf0/Connector/R2020b\"],\"version\":\"1.0\"}"
  Pipe6_3 : Subsystem  ReferencedSubsystem=PipeSubsystemWithMask  lengthPipe=0.36667  areaPipe=3.1416e-06  diaPipe=0.002  directionPipe=right
      settings: PortSchema="{\"entries\":[{\"content\":{\"sides\":[{\"content\":{\"connectorIds\":[\"LConn1\"]},\"type\":\"ConnectorPlacement.EquallySpacedRectSide\",\"uuid\":\"fe1e9e2d-1739-4737-8ec3-440461fb646e\"},{\"content\":{\"connectorIds\":[\"RConn1\"],\"side\":\"RIGHT\"},\"type\":\"ConnectorPlacement.EquallySpacedRectSide\",\"uuid\":\"c44e4257-eb38-4c5c-b0bd-b7832920e0b4\"},{\"content\":{\"connectorIds\":[\"LConn2\"],\"side\":\"TOP\"},\"type\":\"ConnectorPlacement.EquallySpacedRectSide\",\"uuid\":\"152ce001-782f-4a48-bd0b-9533b0313205\"}]},\"type\":\"ConnectorPlacement.EquallySpacedConnector\",\"uuid\":\"fea8adfe-ce64-4d7f-ba34-bc1e0cac7b5f\"}],\"packageUris\":[\"http://schema.mathworks.com/mf0/Connector/R2020b\"],\"version\":\"1.0\"}"
  Pipe7_1 : Subsystem  ReferencedSubsystem=PipeSubsystemWithMask  lengthPipe=0.36667  areaPipe=3.1416e-06  diaPipe=0.002  directionPipe=right
      settings: PortSchema="{\"entries\":[{\"content\":{\"sides\":[{\"content\":{\"connectorIds\":[\"LConn1\"]},\"type\":\"ConnectorPlacement.EquallySpacedRectSide\",\"uuid\":\"fe1e9e2d-1739-4737-8ec3-440461fb646e\"},{\"content\":{\"connectorIds\":[\"RConn1\"],\"side\":\"RIGHT\"},\"type\":\"ConnectorPlacement.EquallySpacedRectSide\",\"uuid\":\"c44e4257-eb38-4c5c-b0bd-b7832920e0b4\"},{\"content\":{\"connectorIds\":[\"LConn2\"],\"side\":\"TOP\"},\"type\":\"ConnectorPlacement.EquallySpacedRectSide\",\"uuid\":\"152ce001-782f-4a48-bd0b-9533b0313205\"}]},\"type\":\"ConnectorPlacement.EquallySpacedConnector\",\"uuid\":\"fea8adfe-ce64-4d7f-ba34-bc1e0cac7b5f\"}],\"packageUris\":[\"http://schema.mathworks.com/mf0/Connector/R2020b\"],\"version\":\"1.0\"}"
  Pipe7_2 : Subsystem  ReferencedSubsystem=PipeSubsystemWithMask  lengthPipe=0.39167  areaPipe=3.1416e-06  diaPipe=0.002  directionPipe=right
      settings: PortSchema="{\"entries\":[{\"content\":{\"sides\":[{\"content\":{\"connectorIds\":[\"LConn1\"]},\"type\":\"ConnectorPlacement.EquallySpacedRectSide\",\"uuid\":\"fe1e9e2d-1739-4737-8ec3-440461fb646e\"},{\"content\":{\"connectorIds\":[\"RConn1\"],\"side\":\"RIGHT\"},\"type\":\"ConnectorPlacement.EquallySpacedRectSide\",\"uuid\":\"c44e4257-eb38-4c5c-b0bd-b7832920e0b4\"},{\"content\":{\"connectorIds\":[\"LConn2\"],\"side\":\"TOP\"},\"type\":\"ConnectorPlacement.EquallySpacedRectSide\",\"uuid\":\"152ce001-782f-4a48-bd0b-9533b0313205\"}]},\"type\":\"ConnectorPlacement.EquallySpacedConnector\",\"uuid\":\"fea8adfe-ce64-4d7f-ba34-bc1e0cac7b5f\"}],\"packageUris\":[\"http://schema.mathworks.com/mf0/Connector/R2020b\"],\"version\":\"1.0\"}"
  Pipe7_3 : Subsystem  ReferencedSubsystem=PipeSubsystemWithMask  lengthPipe=0.36667  areaPipe=3.1416e-06  diaPipe=0.002  directionPipe=right
      settings: PortSchema="{\"entries\":[{\"content\":{\"sides\":[{\"content\":{\"connectorIds\":[\"LConn1\"]},\"type\":\"ConnectorPlacement.EquallySpacedRectSide\",\"uuid\":\"fe1e9e2d-1739-4737-8ec3-440461fb646e\"},{\"content\":{\"connectorIds\":[\"RConn1\"],\"side\":\"RIGHT\"},\"type\":\"ConnectorPlacement.EquallySpacedRectSide\",\"uuid\":\"c44e4257-eb38-4c5c-b0bd-b7832920e0b4\"},{\"content\":{\"connectorIds\":[\"LConn2\"],\"side\":\"TOP\"},\"type\":\"ConnectorPlacement.EquallySpacedRectSide\",\"uuid\":\"152ce001-782f-4a48-bd0b-9533b0313205\"}]},\"type\":\"ConnectorPlacement.EquallySpacedConnector\",\"uuid\":\"fea8adfe-ce64-4d7f-ba34-bc1e0cac7b5f\"}],\"packageUris\":[\"http://schema.mathworks.com/mf0/Connector/R2020b\"],\"version\":\"1.0\"}"
  Pipe8_1 : Subsystem  ReferencedSubsystem=PipeSubsystemWithMask  lengthPipe=0.36667  areaPipe=3.1416e-06  diaPipe=0.002  directionPipe=right
      settings: PortSchema="{\"entries\":[{\"content\":{\"sides\":[{\"content\":{\"connectorIds\":[\"LConn1\"]},\"type\":\"ConnectorPlacement.EquallySpacedRectSide\",\"uuid\":\"fe1e9e2d-1739-4737-8ec3-440461fb646e\"},{\"content\":{\"connectorIds\":[\"RConn1\"],\"side\":\"RIGHT\"},\"type\":\"ConnectorPlacement.EquallySpacedRectSide\",\"uuid\":\"c44e4257-eb38-4c5c-b0bd-b7832920e0b4\"},{\"content\":{\"connectorIds\":[\"LConn2\"],\"side\":\"TOP\"},\"type\":\"ConnectorPlacement.EquallySpacedRectSide\",\"uuid\":\"152ce001-782f-4a48-bd0b-9533b0313205\"}]},\"type\":\"ConnectorPlacement.EquallySpacedConnector\",\"uuid\":\"fea8adfe-ce64-4d7f-ba34-bc1e0cac7b5f\"}],\"packageUris\":[\"http://schema.mathworks.com/mf0/Connector/R2020b\"],\"version\":\"1.0\"}"
  Pipe8_2 : Subsystem  ReferencedSubsystem=PipeSubsystemWithMask  lengthPipe=0.39167  areaPipe=3.1416e-06  diaPipe=0.002  directionPipe=right
      settings: PortSchema="{\"entries\":[{\"content\":{\"sides\":[{\"content\":{\"connectorIds\":[\"LConn1\"]},\"type\":\"ConnectorPlacement.EquallySpacedRectSide\",\"uuid\":\"fe1e9e2d-1739-4737-8ec3-440461fb646e\"},{\"content\":{\"connectorIds\":[\"RConn1\"],\"side\":\"RIGHT\"},\"type\":\"ConnectorPlacement.EquallySpacedRectSide\",\"uuid\":\"c44e4257-eb38-4c5c-b0bd-b7832920e0b4\"},{\"content\":{\"connectorIds\":[\"LConn2\"],\"side\":\"TOP\"},\"type\":\"ConnectorPlacement.EquallySpacedRectSide\",\"uuid\":\"152ce001-782f-4a48-bd0b-9533b0313205\"}]},\"type\":\"ConnectorPlacement.EquallySpacedConnector\",\"uuid\":\"fea8adfe-ce64-4d7f-ba34-bc1e0cac7b5f\"}],\"packageUris\":[\"http://schema.mathworks.com/mf0/Connector/R2020b\"],\"version\":\"1.0\"}"
  Pipe8_3 : Subsystem  ReferencedSubsystem=PipeSubsystemWithMask  lengthPipe=0.36667  areaPipe=3.1416e-06  diaPipe=0.002  directionPipe=right
      settings: PortSchema="{\"entries\":[{\"content\":{\"sides\":[{\"content\":{\"connectorIds\":[\"LConn1\"]},\"type\":\"ConnectorPlacement.EquallySpacedRectSide\",\"uuid\":\"fe1e9e2d-1739-4737-8ec3-440461fb646e\"},{\"content\":{\"connectorIds\":[\"RConn1\"],\"side\":\"RIGHT\"},\"type\":\"ConnectorPlacement.EquallySpacedRectSide\",\"uuid\":\"c44e4257-eb38-4c5c-b0bd-b7832920e0b4\"},{\"content\":{\"connectorIds\":[\"LConn2\"],\"side\":\"TOP\"},\"type\":\"ConnectorPlacement.EquallySpacedRectSide\",\"uuid\":\"152ce001-782f-4a48-bd0b-9533b0313205\"}]},\"type\":\"ConnectorPlacement.EquallySpacedConnector\",\"uuid\":\"fea8adfe-ce64-4d7f-ba34-bc1e0cac7b5f\"}],\"packageUris\":[\"http://schema.mathworks.com/mf0/Connector/R2020b\"],\"version\":\"1.0\"}"
  Pipe9_1 : Subsystem  ReferencedSubsystem=PipeSubsystemWithMask  lengthPipe=0.36667  areaPipe=3.1416e-06  diaPipe=0.002  directionPipe=right
      settings: PortSchema="{\"entries\":[{\"content\":{\"sides\":[{\"content\":{\"connectorIds\":[\"LConn1\"]},\"type\":\"ConnectorPlacement.EquallySpacedRectSide\",\"uuid\":\"fe1e9e2d-1739-4737-8ec3-440461fb646e\"},{\"content\":{\"connectorIds\":[\"RConn1\"],\"side\":\"RIGHT\"},\"type\":\"ConnectorPlacement.EquallySpacedRectSide\",\"uuid\":\"c44e4257-eb38-4c5c-b0bd-b7832920e0b4\"},{\"content\":{\"connectorIds\":[\"LConn2\"],\"side\":\"TOP\"},\"type\":\"ConnectorPlacement.EquallySpacedRectSide\",\"uuid\":\"152ce001-782f-4a48-bd0b-9533b0313205\"}]},\"type\":\"ConnectorPlacement.EquallySpacedConnector\",\"uuid\":\"fea8adfe-ce64-4d7f-ba34-bc1e0cac7b5f\"}],\"packageUris\":[\"http://schema.mathworks.com/mf0/Connector/R2020b\"],\"version\":\"1.0\"}"
  Pipe9_2 : Subsystem  ReferencedSubsystem=PipeSubsystemWithMask  lengthPipe=0.39167  areaPipe=3.1416e-06  diaPipe=0.002  directionPipe=right
      settings: PortSchema="{\"entries\":[{\"content\":{\"sides\":[{\"content\":{\"connectorIds\":[\"LConn1\"]},\"type\":\"ConnectorPlacement.EquallySpacedRectSide\",\"uuid\":\"fe1e9e2d-1739-4737-8ec3-440461fb646e\"},{\"content\":{\"connectorIds\":[\"RConn1\"],\"side\":\"RIGHT\"},\"type\":\"ConnectorPlacement.EquallySpacedRectSide\",\"uuid\":\"c44e4257-eb38-4c5c-b0bd-b7832920e0b4\"},{\"content\":{\"connectorIds\":[\"LConn2\"],\"side\":\"TOP\"},\"type\":\"ConnectorPlacement.EquallySpacedRectSide\",\"uuid\":\"152ce001-782f-4a48-bd0b-9533b0313205\"}]},\"type\":\"ConnectorPlacement.EquallySpacedConnector\",\"uuid\":\"fea8adfe-ce64-4d7f-ba34-bc1e0cac7b5f\"}],\"packageUris\":[\"http://schema.mathworks.com/mf0/Connector/R2020b\"],\"version\":\"1.0\"}"
  Pipe9_3 : Subsystem  ReferencedSubsystem=PipeSubsystemWithMask  lengthPipe=0.36667  areaPipe=3.1416e-06  diaPipe=0.002  directionPipe=right
      settings: PortSchema="{\"entries\":[{\"content\":{\"sides\":[{\"content\":{\"connectorIds\":[\"LConn1\"]},\"type\":\"ConnectorPlacement.EquallySpacedRectSide\",\"uuid\":\"fe1e9e2d-1739-4737-8ec3-440461fb646e\"},{\"content\":{\"connectorIds\":[\"RConn1\"],\"side\":\"RIGHT\"},\"type\":\"ConnectorPlacement.EquallySpacedRectSide\",\"uuid\":\"c44e4257-eb38-4c5c-b0bd-b7832920e0b4\"},{\"content\":{\"connectorIds\":[\"LConn2\"],\"side\":\"TOP\"},\"type\":\"ConnectorPlacement.EquallySpacedRectSide\",\"uuid\":\"152ce001-782f-4a48-bd0b-9533b0313205\"}]},\"type\":\"ConnectorPlacement.EquallySpacedConnector\",\"uuid\":\"fea8adfe-ce64-4d7f-ba34-bc1e0cac7b5f\"}],\"packageUris\":[\"http://schema.mathworks.com/mf0/Connector/R2020b\"],\"version\":\"1.0\"}"
  fluid_in : PMIOPort  Side=Left
  fluid_out : PMIOPort  Port=2  Side=Right
  H : PMIOPort  Port=3  Side=Left
  connections:
  Array Connection/RConn1 -- H/RConn1
  H_39_1_bus/LConn1 -- Array Connection/LConn77
  Bend2_1/RConn1 -- H_39_1/LConn1
  H_38_1_bus/LConn1 -- Array Connection/LConn76
  Bend1_1/RConn1 -- H_38_1/LConn1
  H_37_1_bus/LConn1 -- Array Connection/LConn75
  Pipe37_1/LConn2 -- H_37_1/LConn1
  H_36_2_bus/LConn1 -- Array Connection/LConn74
  Pipe36_2/LConn2 -- H_36_2/LConn1
  H_36_1_bus/LConn1 -- Array Connection/LConn73
  Pipe36_1/LConn2 -- H_36_1/LConn1
  Pipe36_1/RConn1 -- Pipe36_2/LConn1
  H_35_2_bus/LConn1 -- Array Connection/LConn72
  Pipe35_2/LConn2 -- H_35_2/LConn1
  H_35_1_bus/LConn1 -- Array Connection/LConn71
  Pipe35_1/LConn2 -- H_35_1/LConn1
  Pipe35_1/RConn1 -- Pipe35_2/LConn1
  H_34_1_bus/LConn1 -- Array Connection/LConn70
  Pipe34_1/LConn2 -- H_34_1/LConn1
  H_33_2_bus/LConn1 -- Array Connection/LConn69
  Pipe33_2/LConn2 -- H_33_2/LConn1
  H_33_1_bus/LConn1 -- Array Connection/LConn68
  Pipe33_1/LConn2 -- H_33_1/LConn1
  Pipe33_1/RConn1 -- Pipe33_2/LConn1
  H_32_1_bus/LConn1 -- Array Connection/LConn67
  Pipe32_1/LConn2 -- H_32_1/LConn1
  H_31_1_bus/LConn1 -- Array Connection/LConn66
  Pipe31_1/LConn2 -- H_31_1/LConn1
  H_30_2_bus/LConn1 -- Array Connection/LConn65
  Pipe30_2/LConn2 -- H_30_2/LConn1
  H_30_1_bus/LConn1 -- Array Connection/LConn64
  Pipe30_1/LConn2 -- H_30_1/LConn1
  Pipe30_1/RConn1 -- Pipe30_2/LConn1
  H_29_1_bus/LConn1 -- Array Connection/LConn63
  Pipe29_1/LConn2 -- H_29_1/LConn1
  H_28_2_bus/LConn1 -- Array Connection/LConn62
  Pipe28_2/LConn2 -- H_28_2/LConn1
  H_28_1_bus/LConn1 -- Array Connection/LConn61
  Pipe28_1/LConn2 -- H_28_1/LConn1
  Pipe28_1/RConn1 -- Pipe28_2/LConn1
  H_27_2_bus/LConn1 -- Array Connection/LConn60
  Pipe27_2/LConn2 -- H_27_2/LConn1
  H_27_1_bus/LConn1 -- Array Connection/LConn59
  Pipe27_1/LConn2 -- H_27_1/LConn1
  Pipe27_1/RConn1 -- Pipe27_2/LConn1
  Pipe26_1/LConn1 -- Bend2_1/LConn2
  H_26_1_bus/LConn1 -- Array Connection/LConn58
  Pipe26_1/LConn2 -- H_26_1/LConn1
  Pipe25_1/RConn1 -- Bend1_1/LConn1
  H_25_1_bus/LConn1 -- Array Connection/LConn57
  Pipe25_1/LConn2 -- H_25_1/LConn1
  H_24_2_bus/LConn1 -- Array Connection/LConn56
  Pipe24_2/LConn2 -- H_24_2/LConn1
  H_24_1_bus/LConn1 -- Array Connection/LConn55
  Pipe24_1/LConn2 -- H_24_1/LConn1
  Pipe24_1/RConn1 -- Pipe24_2/LConn1
  H_23_2_bus/LConn1 -- Array Connection/LConn54
  Pipe23_2/LConn2 -- H_23_2/LConn1
  H_23_1_bus/LConn1 -- Array Connection/LConn53
  Pipe23_1/LConn2 -- H_23_1/LConn1
  Pipe23_1/RConn1 -- Pipe23_2/LConn1
  H_22_1_bus/LConn1 -- Array Connection/LConn52
  Pipe22_1/LConn2 -- H_22_1/LConn1
  H_21_2_bus/LConn1 -- Array Connection/LConn51
  Pipe21_2/LConn2 -- H_21_2/LConn1
  H_21_1_bus/LConn1 -- Array Connection/LConn50
  Pipe21_1/LConn2 -- H_21_1/LConn1
  Pipe21_1/RConn1 -- Pipe21_2/LConn1
  H_20_1_bus/LConn1 -- Array Connection/LConn49
  Pipe20_1/LConn2 -- H_20_1/LConn1
  H_19_1_bus/LConn1 -- Array Connection/LConn48
  Pipe19_1/LConn2 -- H_19_1/LConn1
  H_18_2_bus/LConn1 -- Array Connection/LConn47
  Pipe18_2/LConn2 -- H_18_2/LConn1
  H_18_1_bus/LConn1 -- Array Connection/LConn46
  Pipe18_1/LConn2 -- H_18_1/LConn1
  Pipe18_1/RConn1 -- Pipe18_2/LConn1
  H_17_1_bus/LConn1 -- Array Connection/LConn45
  Pipe17_1/LConn2 -- H_17_1/LConn1
  H_16_2_bus/LConn1 -- Array Connection/LConn44
  Pipe16_2/LConn2 -- H_16_2/LConn1
  H_16_1_bus/LConn1 -- Array Connection/LConn43
  Pipe16_1/LConn2 -- H_16_1/LConn1
  Pipe16_1/RConn1 -- Pipe16_2/LConn1
  H_15_2_bus/LConn1 -- Array Connection/LConn42
  Pipe15_2/LConn2 -- H_15_2/LConn1
  H_15_1_bus/LConn1 -- Array Connection/LConn41
  Pipe15_1/LConn2 -- H_15_1/LConn1
  Pipe15_1/RConn1 -- Pipe15_2/LConn1
  H_14_1_bus/LConn1 -- Array Connection/LConn40
  Pipe14_1/LConn2 -- H_14_1/LConn1
  Pipe13_1/LConn1 -- Bend1_1/LConn2
  Pipe37_1/RConn1 -- Pipe13_3/RConn1 -- fluid_out/RConn1
  H_13_3_bus/LConn1 -- Array Connection/LConn39
  Pipe13_3/LConn2 -- H_13_3/LConn1
  H_13_2_bus/LConn1 -- Array Connection/LConn38
  Pipe13_2/LConn2 -- H_13_2/LConn1
  H_13_1_bus/LConn1 -- Array Connection/LConn37
  Pipe13_1/LConn2 -- H_13_1/LConn1
  Pipe13_2/RConn1 -- Pipe13_3/LConn1
  Pipe13_1/RConn1 -- Pipe13_2/LConn1
  Pipe12_1/LConn1 -- Pipe25_1/LConn1 -- Pipe24_2/RConn1
  Pipe36_2/RConn1 -- Pipe12_3/RConn1 -- Pipe37_1/LConn1
  H_12_3_bus/LConn1 -- Array Connection/LConn36
  Pipe12_3/LConn2 -- H_12_3/LConn1
  H_12_2_bus/LConn1 -- Array Connection/LConn35
  Pipe12_2/LConn2 -- H_12_2/LConn1
  H_12_1_bus/LConn1 -- Array Connection/LConn34
  Pipe12_1/LConn2 -- H_12_1/LConn1
  Pipe12_2/RConn1 -- Pipe12_3/LConn1
  Pipe12_1/RConn1 -- Pipe12_2/LConn1
  Pipe11_1/LConn1 -- Pipe24_1/LConn1 -- Pipe23_2/RConn1
  Pipe35_2/RConn1 -- Pipe11_3/RConn1 -- Pipe36_1/LConn1
  H_11_3_bus/LConn1 -- Array Connection/LConn33
  Pipe11_3/LConn2 -- H_11_3/LConn1
  H_11_2_bus/LConn1 -- Array Connection/LConn32
  Pipe11_2/LConn2 -- H_11_2/LConn1
  H_11_1_bus/LConn1 -- Array Connection/LConn31
  Pipe11_1/LConn2 -- H_11_1/LConn1
  Pipe11_2/RConn1 -- Pipe11_3/LConn1
  Pipe11_1/RConn1 -- Pipe11_2/LConn1
  Pipe10_1/LConn1 -- Pipe23_1/LConn1 -- Pipe22_1/RConn1
  Pipe34_1/RConn1 -- Pipe10_3/RConn1 -- Pipe35_1/LConn1
  H_10_3_bus/LConn1 -- Array Connection/LConn30
  Pipe10_3/LConn2 -- H_10_3/LConn1
  H_10_2_bus/LConn1 -- Array Connection/LConn29
  Pipe10_2/LConn2 -- H_10_2/LConn1
  H_10_1_bus/LConn1 -- Array Connection/LConn28
  Pipe10_1/LConn2 -- H_10_1/LConn1
  Pipe10_2/RConn1 -- Pipe10_3/LConn1
  Pipe10_1/RConn1 -- Pipe10_2/LConn1
  Pipe9_1/LConn1 -- Pipe22_1/LConn1 -- Pipe21_2/RConn1
  Pipe33_2/RConn1 -- Pipe9_3/RConn1 -- Pipe34_1/LConn1
  H_9_3_bus/LConn1 -- Array Connection/LConn27
  Pipe9_3/LConn2 -- H_9_3/LConn1
  H_9_2_bus/LConn1 -- Array Connection/LConn26
  Pipe9_2/LConn2 -- H_9_2/LConn1
  H_9_1_bus/LConn1 -- Array Connection/LConn25
  Pipe9_1/LConn2 -- H_9_1/LConn1
  Pipe9_2/RConn1 -- Pipe9_3/LConn1
  Pipe9_1/RConn1 -- Pipe9_2/LConn1
  Pipe8_1/LConn1 -- Pipe21_1/LConn1 -- Pipe20_1/RConn1
  Pipe32_1/RConn1 -- Pipe8_3/RConn1 -- Pipe33_1/LConn1
  H_8_3_bus/LConn1 -- Array Connection/LConn24
  Pipe8_3/LConn2 -- H_8_3/LConn1
  H_8_2_bus/LConn1 -- Array Connection/LConn23
  Pipe8_2/LConn2 -- H_8_2/LConn1
  H_8_1_bus/LConn1 -- Array Connection/LConn22
  Pipe8_1/LConn2 -- H_8_1/LConn1
  Pipe8_2/RConn1 -- Pipe8_3/LConn1
  Pipe8_1/RConn1 -- Pipe8_2/LConn1
  Pipe7_1/LConn1 -- Pipe20_1/LConn1 -- Pipe19_1/RConn1
  Pipe31_1/RConn1 -- Pipe7_3/RConn1 -- Pipe32_1/LConn1
  H_7_3_bus/LConn1 -- Array Connection/LConn21
  Pipe7_3/LConn2 -- H_7_3/LConn1
  H_7_2_bus/LConn1 -- Array Connection/LConn20
  Pipe7_2/LConn2 -- H_7_2/LConn1
  H_7_1_bus/LConn1 -- Array Connection/LConn19
  Pipe7_1/LConn2 -- H_7_1/LConn1
  Pipe7_2/RConn1 -- Pipe7_3/LConn1
  Pipe7_1/RConn1 -- Pipe7_2/LConn1
  Pipe6_1/LConn1 -- Pipe19_1/LConn1 -- Pipe18_2/RConn1
  Pipe30_2/RConn1 -- Pipe6_3/RConn1 -- Pipe31_1/LConn1
  H_6_3_bus/LConn1 -- Array Connection/LConn18
  Pipe6_3/LConn2 -- H_6_3/LConn1
  H_6_2_bus/LConn1 -- Array Connection/LConn17
  Pipe6_2/LConn2 -- H_6_2/LConn1
  H_6_1_bus/LConn1 -- Array Connection/LConn16
  Pipe6_1/LConn2 -- H_6_1/LConn1
  Pipe6_2/RConn1 -- Pipe6_3/LConn1
  Pipe6_1/RConn1 -- Pipe6_2/LConn1
  Pipe5_1/LConn1 -- Pipe18_1/LConn1 -- Pipe17_1/RConn1
  Pipe29_1/RConn1 -- Pipe5_3/RConn1 -- Pipe30_1/LConn1
  H_5_3_bus/LConn1 -- Array Connection/LConn15
  Pipe5_3/LConn2 -- H_5_3/LConn1
  H_5_2_bus/LConn1 -- Array Connection/LConn14
  Pipe5_2/LConn2 -- H_5_2/LConn1
  H_5_1_bus/LConn1 -- Array Connection/LConn13
  Pipe5_1/LConn2 -- H_5_1/LConn1
  Pipe5_2/RConn1 -- Pipe5_3/LConn1
  Pipe5_1/RConn1 -- Pipe5_2/LConn1
  Pipe4_1/LConn1 -- Pipe17_1/LConn1 -- Pipe16_2/RConn1
  Pipe28_2/RConn1 -- Pipe4_3/RConn1 -- Pipe29_1/LConn1
  H_4_3_bus/LConn1 -- Array Connection/LConn12
  Pipe4_3/LConn2 -- H_4_3/LConn1
  H_4_2_bus/LConn1 -- Array Connection/LConn11
  Pipe4_2/LConn2 -- H_4_2/LConn1
  H_4_1_bus/LConn1 -- Array Connection/LConn10
  Pipe4_1/LConn2 -- H_4_1/LConn1
  Pipe4_2/RConn1 -- Pipe4_3/LConn1
  Pipe4_1/RConn1 -- Pipe4_2/LConn1
  Pipe3_1/LConn1 -- Pipe16_1/LConn1 -- Pipe15_2/RConn1
  Pipe27_2/RConn1 -- Pipe3_3/RConn1 -- Pipe28_1/LConn1
  H_3_3_bus/LConn1 -- Array Connection/LConn9
  Pipe3_3/LConn2 -- H_3_3/LConn1
  H_3_2_bus/LConn1 -- Array Connection/LConn8
  Pipe3_2/LConn2 -- H_3_2/LConn1
  H_3_1_bus/LConn1 -- Array Connection/LConn7
  Pipe3_1/LConn2 -- H_3_1/LConn1
  Pipe3_2/RConn1 -- Pipe3_3/LConn1
  Pipe3_1/RConn1 -- Pipe3_2/LConn1
  Pipe2_1/LConn1 -- Pipe15_1/LConn1 -- Pipe14_1/RConn1
  Pipe26_1/RConn1 -- Pipe2_3/RConn1 -- Pipe27_1/LConn1
  H_2_3_bus/LConn1 -- Array Connection/LConn6
  Pipe2_3/LConn2 -- H_2_3/LConn1
  H_2_2_bus/LConn1 -- Array Connection/LConn5
  Pipe2_2/LConn2 -- H_2_2/LConn1
  H_2_1_bus/LConn1 -- Array Connection/LConn4
  Pipe2_1/LConn2 -- H_2_1/LConn1
  Pipe2_2/RConn1 -- Pipe2_3/LConn1
  Pipe2_1/RConn1 -- Pipe2_2/LConn1
  Pipe14_1/LConn1 -- Pipe1_1/LConn1 -- fluid_in/RConn1
  Pipe1_3/RConn1 -- Bend2_1/LConn1
  H_1_3_bus/LConn1 -- Array Connection/LConn3
  Pipe1_3/LConn2 -- H_1_3/LConn1
  H_1_2_bus/LConn1 -- Array Connection/LConn2
  Pipe1_2/LConn2 -- H_1_2/LConn1
  H_1_1_bus/LConn1 -- Array Connection/LConn1
  Pipe1_1/LConn2 -- H_1_1/LConn1
  Pipe1_2/RConn1 -- Pipe1_3/LConn1
  Pipe1_1/RConn1 -- Pipe1_2/LConn1
